simulink model "LunarMicrogrid_Full"  (R2026b)
settings: Solver=ode23t  StopTime=simulation.timeSim  MaxStep=1/(5*solarPlant.converterSwitchingFrequency)  AbsTol=1e-3
PreLoadFcn:
  | run('LunarMicrogridA_Data');
values from neighbouring files (symbols this model uses):
  Csc = Csc_cell/Ns_sc*Np_sc    (= 200)    [LunarDAB_Params.m]
  eta_sc = 0.95    [LunarDAB_Params.m]
  fsw = 100e3    (= 100000)    [LunarDAB_Params.m]
  k_restore = 1    [LunarDAB_Params.m]
  kiCurrent = 2    [LunarDAB_Params.m]
  kiVoltage = 8    [LunarDAB_Params.m]
  kpCurrent = 0.005    [LunarDAB_Params.m]
  kpVoltage = 0.4    [LunarDAB_Params.m]
  lTotal = lSeries + Llk    [LunarDAB_Params.m]
  P170_dt = 1e-4    (= 0.0001)    [P170_PV_Initialize.m]
  P170_Imp = im(ix)    [P170_PV_Initialize.m]
  P170_Vmp = vm(ix)    [P170_PV_Initialize.m]
  Rd_bat = dV_droop/Ibat_max    (= 0.232258064516)    [LunarDAB_Params.m]
  SC_enable = 1    [LunarDAB_Params.m]
  thetaIC = 0    [LunarDAB_Params.m]
  thetaMaxDab = pi/4    (= 0.785398163397)    [LunarDAB_Params.m]
  Tsw = 1/fsw    (= 1e-05)    [LunarDAB_Params.m]
  Vsc0 = sqrt((Vsc_max^2 + Vsc_min^2)/2)    [LunarDAB_Params.m]
  Vsc_max = 119    [LunarDAB_Params.m]
  Vsc_min = 66    [LunarDAB_Params.m]
undefined symbols (not defined in the file or in its folder): a_lpf_sys, battery, bms, connectedLoad, dcVoltage, DiscIntNeverNeededParam, eta_dab, Ibat_sign, mmc, Ndab, P170_T, pvDroop, sc, sensor, socLimit, solarPlant
libraries: sl_discontinuities x13, fl_lib x13, nesl_utility x13, simulink x7, batteryecm_lib x1, simulink_extras x1, ee_lib x1
(part 2 of 8)

== system LunarMicrogrid_Full/BESS Controller ==
  note: Current_Controller
  note: Voltage Controller
  Vref : Inport
  I_V1 : Inport  Port=2
  Vout : Inport  Port=3
  DABCtrl2 : Subsystem  AncestorBlock=mcblib/Control/Synchronous Machine/Controllers/PI Controller  mask(PID 1dof){Controller=PI, Form=Parallel, TimeDomain=Discrete-time, UseExternalTs=off, SampleTime=Tsw, IntegratorMethod=Forward Euler, FilterMethod=Forward Euler, ControllerParametersSource=internal, P=kpCurrent, I=kiCurrent, UseKiTs=off, D=0, UseExternalDerivativeSource=off, N=100, UseFilter=on, TunerSelectOption=Transfer Function Based (PID Tuner App), ZeroCross=on, InitialConditionSource=internal, InitialConditionForIntegrator=thetaIC, InitialConditionForFilter=0, DifferentiatorICPrevScaledInput=0, ExternalReset=none, IgnoreLimit=off, TrackingMode=off, Kt=1, LimitOutput=on, SatLimitsSource=external, UpperSaturationLimit=thetaMaxDab, LowerSaturationLimit=-thetaMaxDab, LinearizeAsGain=off, AntiWindupMode=clamping, Kb=1, LimitIntegrator=off, UpperIntegratorSaturationLimit=inf, LowerIntegratorSaturationLimit=-inf, RndMeth=Simplest, SaturateOnIntegerOverflow=off, LockScale=off, PGainOutDataTypeStr=Inherit: Same as input, PProdOutDataTypeStr=Inherit: Same as first input, POutMin=[], POutMax=[], IGainOutDataTypeStr=Inherit: Same as input, IProdOutDataTypeStr=Inherit: Same as first input, IOutMin=[], IOutMax=[], DGainOutDataTypeStr=Inherit: Inherit via internal rule, DProdOutDataTypeStr=Inherit: Inherit via internal rule, DOutMin=[], DOutMax=[], NGainOutDataTypeStr=Inherit: Inherit via internal rule, NProdOutDataTypeStr=Inherit: Inherit via internal rule, NOutMin=[], NOutMax=[], SumOutDataTypeStr=Inherit: Same as first input, SumOutMin=[], SumOutMax=[], SaturationOutDataTypeStr=Inherit: Inherit via back propagation, SaturationOutMin=[], SaturationOutMax=[], PParamDataTypeStr=Inherit: Inherit via internal rule, PParamMin=[], PParamMax=[], IParamDataTypeStr=Inherit: Inherit via internal rule, IParamMin=[], IParamMax=[], DParamDataTypeStr=Inherit: Inherit via internal rule, DParamMin=[], DParamMax=[], NParamDataTypeStr=Inherit: Inherit via internal rule, NParamMin=[], NParamMax=[], KbParamDataTypeStr=Inherit: Inherit via internal rule, KbParamMin=[], KbParamMax=[], KtParamDataTypeStr=Inherit: Inherit via internal rule, KtParamMin=[], KtParamMax=[], KbOutDataTypeStr=Inherit: Inherit via internal rule, KbOutMin=[], KbOutMax=[], KtOutDataTypeStr=Inherit: Inherit via internal rule, KtOutMin=[], KtOutMax=[], IntegratorOutDataTypeStr=Inherit: Inherit via internal rule, IntegratorOutMin=[], IntegratorOutMax=[], FilterOutDataTypeStr=Inherit: Inherit via internal rule, FilterOutMin=[], FilterOutMax=[], SumI1OutDataTypeStr=Inherit: Inherit via internal rule, SumI1OutMin=[], SumI1OutMax=[], SumI2OutDataTypeStr=Inherit: Inherit via internal rule, SumI2OutMin=[], SumI2OutMax=[], SumI3OutDataTypeStr=Inherit: Inherit via internal rule, SumI3OutMin=[], SumI3OutMax=[], SumI4OutDataTypeStr=Inherit: Inherit via internal rule, SumI4OutMin=[], SumI4OutMax=[], SumDOutDataTypeStr=Inherit: Inherit via internal rule, SumDOutMin=[], SumDOutMax=[], SumAccumDataTypeStr=Inherit: Inherit via internal rule, SumI1AccumDataTypeStr=Inherit: Inherit via internal rule, SumI2AccumDataTypeStr=Inherit: Inherit via internal rule, SumI3AccumDataTypeStr=Inherit: Inherit via internal rule, SumI4AccumDataTypeStr=Inherit: Inherit via internal rule, SumDAccumDataTypeStr=Inherit: Inherit via internal rule, DifferentiatorOutDataTypeStr=Inherit: Inherit via internal rule, DifferentiatorOutMin=[], DifferentiatorOutMax=[], FilterDiffNumProductOutputDataTypeStr=Inherit: Inherit via internal rule, FilterDiffDenProductOutputDataTypeStr=Inherit: Inherit via internal rule, FilterDiffNumAccumDataTypeStr=Inherit: Inherit via internal rule, FilterDiffDenAccumDataTypeStr=Inherit: Inherit via internal rule, FilterDiffOutCoefDataTypeStr=Inherit: Inherit via internal rule, FilterDiffOutCoefMin=[], FilterDiffOutCoefMax=[], ReciprocalOutDataTypeStr=Inherit: Inherit via internal rule, ReciprocalOutMin=[], ReciprocalOutMax=[], SumDenOutDataTypeStr=Inherit: Inherit via internal rule, SumDenOutMin=[], SumDenOutMax=[], SumNumOutDataTypeStr=Inherit: Inherit via internal rule, SumNumOutMin=[], SumNumOutMax=[], SumDenAccumDataTypeStr=Inherit: Inherit via internal rule, SumNumAccumDataTypeStr=Inherit: Inherit via internal rule, DivideOutDataTypeStr=Inherit: Inherit via internal rule, DivideOutMin=[], DivideOutMax=[], UdiffTsProdOutDataTypeStr=Inherit: Inherit via internal rule, UdiffTsProdOutMin=[], UdiffTsProdOutMax=[], NTsProdOutDataTypeStr=Inherit: Inherit via internal rule, NTsProdOutMin=[], NTsProdOutMax=[], UintegralTsProdOutDataTypeStr=Inherit: Inherit via internal rule, UintegralTsProdOutMin=[], UintegralTsProdOutMax=[], UngainTsProdOutDataTypeStr=Inherit: Inherit via internal rule, UngainTsProdOutMin=[], UngainTsProdOutMax=[], ClampingZeroOutDataTypeStr=Inherit: Inherit via back propagation, ClampingZeroOutMin=[], ClampingZeroOutMax=[], FilterDenConstantOutDataTypeStr=Inherit: Inherit via back propagation, FilterDenConstantOutMin=[], FilterDenConstantOutMax=[], PCopyOutDataTypeStr=Inherit: Inherit via back propagation, PCopyOutMin=[], PCopyOutMax=[], NCopyOutDataTypeStr=Inherit: Inherit via back propagation, NCopyOutMin=[], NCopyOutMax=[], IntegratorContinuousStateAttributes='', IntegratorStateIdentifier=, IntegratorStateMustResolveToSignalObject=off, IntegratorRTWStateStorageClass=Auto, IntegratorRTWStateStorageTypeQualifier=, FilterContinuousStateAttributes='', FilterStateIdentifier=, FilterStateMustResolveToSignalObject=off, FilterRTWStateStorageClass=Auto, FilterRTWStateStorageTypeQualifier=, ParallelPVariant=InternalParameters, IdealPVariant=Disabled, IVariant=InternalParameters, DVariant=Disabled, IntegratorVariant=Discrete, SatVariant=External, AWVariant=DiscClampingParallel, PCopyVariant=Disabled, TRVariant=Disabled, FdbkBlocksVariant=Forward, IdealPFdbkVariant=Disabled, SatFdbkVariant=Disabled, DerivativeFilterVariant=Disabled, NVariant=Disabled, NCopyVariant=Disabled_SignalSpec, FilterICVariant=Disabled, IntegratorICVariant=InternalICs, ExternalResetVariant=Disabled, TRSumVariant=Passthrough, SumFdbkVariant=Disabled, SumVariant=Sum_PI, TsampFilterVariant=InternalTs, TsampNgainVariant=Passthrough, TsampIntegralVariant=Disabled_SignalSpec, ExternalSaturationOutDataTypeStr=Inherit: Same as second input, DerivativeSourceVariant=Disabled, InitialConditionSetting=Auto, PreIntVariant=InternalPreInt}
      mask prompts: Controller "Simulink:masks:Controller_MP"; Form "Simulink:masks:Form_MP"; TimeDomain "Simulink:masks:TimeDomain_MP"; UseExternalTs "Simulink:masks:PIDBlockInTriggeredSubsystem_MP"; SampleTime "Simulink:masks:SampleTime1ForInherited_MP"; IntegratorMethod "Simulink:masks:IntegratorMethod_MP"; FilterMethod "Simulink:masks:FilterMethod_MP"; ControllerParametersSource "Simulink:masks:Source_MP"; P "Simulink:masks:ProportionalP_MP"; I "Simulink:masks:IntegralI_MP"; UseKiTs "Simulink:masks:UseITs_MP"; D "Simulink:masks:DerivativeD_MP"; UseExternalDerivativeSource "Simulink:masks:UseExternalDerivative_MP"; N "Simulink:masks:FilterCoefficientN_MP"; UseFilter "Simulink:masks:UseFilter_MP"; TunerSelectOption "Simulink:masks:PIDAutoTuningMethodSelect_MP"; ZeroCross "Simulink:masks:EnableZerocrossingDetection_MP"; InitialConditionSource "Simulink:masks:Source_MP"; InitialConditionForIntegrator "Simulink:masks:Integrator_MP"; InitialConditionForFilter "Simulink:masks:Filter_MP"; DifferentiatorICPrevScaledInput "Simulink:masks:Differentiator_MP"; ExternalReset "Simulink:masks:ExternalReset_MP"; IgnoreLimit "Simulink:masks:IgnoreResetWhenLinearizing_MP"; TrackingMode "Simulink:masks:EnableTrackingMode_MP"; Kt "Simulink:masks:TrackingCoefficientKt_MP"; LimitOutput "Simulink:masks:LimitOutput_MP"; SatLimitsSource "Simulink:masks:Source_MP"; UpperSaturationLimit "Simulink:masks:UpperSaturationLimit_MP"; LowerSaturationLimit "Simulink:masks:LowerSaturationLimit_MP"; LinearizeAsGain "Simulink:masks:IgnoreSaturationWhenLinearizing_MP"; AntiWindupMode "Simulink:masks:AntiwindupMethod_MP"; Kb "Simulink:masks:BackcalculationCoefficientKb_MP"; LimitIntegrator "Simulink:blkprm_prompts:IntegratorLimitOutput"; UpperIntegratorSaturationLimit "Simulink:masks:UpperSaturationLimit_MP"; LowerIntegratorSaturationLimit "Simulink:masks:LowerSaturationLimit_MP"; RndMeth "Simulink:masks:IntegerRoundingMode_MP"; SaturateOnIntegerOverflow "Simulink:masks:SaturateOnIntegerOverflow_MP"; LockScale "Simulink:masks:LockDataTypeAgainstFxpTools_MP"; PGainOutDataTypeStr "Simulink:masks:PProductOutput_MP"; PProdOutDataTypeStr "Simulink:masks:PProductOutput_MP"; IGainOutDataTypeStr "Simulink:masks:IProductOutput_MP"; IProdOutDataTypeStr "Simulink:masks:IProductOutput_MP"; DGainOutDataTypeStr "Simulink:masks:DProductOutput_MP"; DProdOutDataTypeStr "Simulink:masks:DProductOutput_MP"; NGainOutDataTypeStr "Simulink:masks:NProductOutput_MP"; NProdOutDataTypeStr "Simulink:masks:NProductOutput_MP"; SumOutDataTypeStr "Simulink:masks:SumOutput_MP"; SaturationOutDataTypeStr "Simulink:masks:SaturationOutput_MP"; PParamDataTypeStr "Simulink:masks:PParameter_MP"; IParamDataTypeStr "Simulink:masks:IParameter_MP"; DParamDataTypeStr "Simulink:masks:DParameter_MP"; NParamDataTypeStr "Simulink:masks:NParameter_MP"; KbParamDataTypeStr "Simulink:masks:KbParameter_MP"; KtParamDataTypeStr "Simulink:masks:KtParameter_MP"; KbOutDataTypeStr "Simulink:masks:KbProductOutput_MP"; KtOutDataTypeStr "Simulink:masks:KtProductOutput_MP"; IntegratorOutDataTypeStr "Simulink:masks:IntegratorOutput_MP"; FilterOutDataTypeStr "Simulink:masks:FilterOutput_MP"; SumI1OutDataTypeStr "Simulink:masks:SumI1Output_MP"; SumI2OutDataTypeStr "Simulink:masks:SumI2Output_MP"; SumI3OutDataTypeStr "Simulink:masks:SumI3Output_MP"; SumI4OutDataTypeStr "Simulink:masks:SumI4Output_MP"; SumDOutDataTypeStr "Simulink:masks:SumDOutput_MP"; SumAccumDataTypeStr "Simulink:masks:AccumulatorOfSum_MP"; SumI1AccumDataTypeStr "Simulink:masks:AccumulatorOfSumI1_MP"; SumI2AccumDataTypeStr "Simulink:masks:AccumulatorOfSumI2_MP"; SumI3AccumDataTypeStr "Simulink:masks:AccumulatorOfSumI3_MP"; SumI4AccumDataTypeStr "Simulink:masks:AccumulatorOfSumI4_MP"; SumDAccumDataTypeStr "Simulink:masks:AccumulatorOfSumD_MP"; DifferentiatorOutDataTypeStr "Simulink:masks:DifferentiatorOutput_MP"; FilterDiffNumProductOutputDataTypeStr "Simulink:masks:FilterDiffNumProductOutput_MP"; FilterDiffDenProductOutputDataTypeStr "Simulink:masks:FilterDiffDenProductOutput_MP"; FilterDiffNumAccumDataTypeStr "Simulink:masks:FilterDiffNumAccumulator_MP"; FilterDiffDenAccumDataTypeStr "Simulink:masks:FilterDiffDenAccumulator_MP"; FilterDiffOutCoefDataTypeStr "Simulink:masks:FilterDiffCoefficientOutput_MP"; ReciprocalOutDataTypeStr "Simulink:masks:FilterDiffReciprocalOutput_MP"; SumDenOutDataTypeStr "Simulink:masks:FilterDiffSumDenOutput_MP"; SumNumOutDataTypeStr "Simulink:masks:FilterDiffSumNumOutput_MP"; SumDenAccumDataTypeStr "Simulink:masks:FilterDiffSumDenAccumulator_MP"; SumNumAccumDataTypeStr "Simulink:masks:FilterDiffSumNumAccumulator_MP"; DivideOutDataTypeStr "Simulink:masks:FilterDiffDivideOutput_MP"; UdiffTsProdOutDataTypeStr "Simulink:masks:UdiffTsProdOut_MP"; NTsProdOutDataTypeStr "Simulink:masks:NTsProdOut_MP"; UintegralTsProdOutDataTypeStr "Simulink:masks:UintegralTsProdOut_MP"; UngainTsProdOutDataTypeStr "Simulink:masks:UngainTsProdOut_MP"; ClampingZeroOutDataTypeStr "Simulink:masks:ClampingAlgorithmConstantZero_MP"; FilterDenConstantOutDataTypeStr "Simulink:masks:FilterCoeffDenConstant_MP"; PCopyOutDataTypeStr "Simulink:masks:PCopyConstant_MP"; NCopyOutDataTypeStr "Simulink:masks:NCopyConstant_MP"; IntegratorContinuousStateAttributes "Simulink:masks:StateNameegposition_MP"; IntegratorStateIdentifier "Simulink:masks:StateName_MP"; IntegratorStateMustResolveToSignalObject "Simulink:masks:StateNameMustResolveToSimulinkSignalObject_MP"; IntegratorRTWStateStorageClass "Simulink:masks:CodeGenerationStorageClass_MP"; IntegratorRTWStateStorageTypeQualifier "Simulink:masks:CodeGenerationStorageTypeQualifier_MP"; FilterContinuousStateAttributes "Simulink:masks:StateNameegposition_MP"; FilterStateIdentifier "Simulink:masks:StateName_MP"; FilterStateMustResolveToSignalObject "Simulink:masks:StateNameMustResolveToSimulinkSignalObject_MP"; FilterRTWStateStorageClass "Simulink:masks:CodeGenerationStorageClass_MP"; FilterRTWStateStorageTypeQualifier "Simulink:masks:CodeGenerationStorageTypeQualifier_MP"; ParallelPVariant "Simulink:blkprm_prompts:OverrideUsingVariant"; IdealPVariant "Simulink:blkprm_prompts:OverrideUsingVariant"; IVariant "Simulink:blkprm_prompts:OverrideUsingVariant"; DVariant "Simulink:blkprm_prompts:OverrideUsingVariant"; IntegratorVariant "Simulink:blkprm_prompts:OverrideUsingVariant"; SatVariant "Simulink:blkprm_prompts:OverrideUsingVariant"; AWVariant "Simulink:blkprm_prompts:OverrideUsingVariant"; PCopyVariant "Simulink:blkprm_prompts:OverrideUsingVariant"; TRVariant "Simulink:blkprm_prompts:OverrideUsingVariant"; FdbkBlocksVariant "Simulink:blkprm_prompts:OverrideUsingVariant"; IdealPFdbkVariant "Simulink:blkprm_prompts:OverrideUsingVariant"; SatFdbkVariant "Simulink:blkprm_prompts:OverrideUsingVariant"; DerivativeFilterVariant "Simulink:blkprm_prompts:OverrideUsingVariant"; NVariant "Simulink:blkprm_prompts:OverrideUsingVariant"; NCopyVariant "Simulink:blkprm_prompts:OverrideUsingVariant"; FilterICVariant "Simulink:blkprm_prompts:OverrideUsingVariant"; IntegratorICVariant "Simulink:blkprm_prompts:OverrideUsingVariant"; ExternalResetVariant "Simulink:blkprm_prompts:OverrideUsingVariant"; TRSumVariant "Simulink:blkprm_prompts:OverrideUsingVariant"; SumFdbkVariant "Simulink:blkprm_prompts:OverrideUsingVariant"; SumVariant "Simulink:blkprm_prompts:OverrideUsingVariant"; TsampFilterVariant "Simulink:Variants:LabelComboBox"; TsampNgainVariant "Simulink:Variants:LabelComboBox"; TsampIntegralVariant "Simulink:Variants:LabelComboBox"; ExternalSaturationOutDataTypeStr "Simulink:masks:SaturationOutput_MP"; DerivativeSourceVariant "Simulink:Variants:LabelComboBox"; InitialConditionSetting "Simulink:blkprm_prompts:IntegratorInitCondSetting"; PreIntVariant "Simulink:Variants:LabelComboBox"
      mask help: Simulink:masks:PID1dof_MD
      mask init:
      | SampleTime = pidpack.PIDConfig.maskInitialization(gcbh, SampleTime);
      settings: LibrarySourceBlock=mcblib/Control/Synchronous Machine/Controllers/PI Controller  DeleteFcn=pidpack.PIDConfig.utilCloseTuner(gcb)  ModelCloseFcn=pidpack.PIDConfig.utilCloseTuner(gcb)  NameChangeFcn=pidpack.PIDConfig.utilUpdateTunerName(gcb)
      mask TypeOptions Controller: Simulink:masks:PID | Simulink:masks:PI | Simulink:masks:PD | Simulink:masks:P | Simulink:masks:I
      mask Callback Controller: pidpack.PIDConfig.callbackMaskVisibilities(gcbh,'UpdateCompFormula')
      mask TypeOptions Form: Simulink:masks:Ideal | Simulink:masks:Parallel
      mask Callback Form: pidpack.PIDConfig.callbackMaskVisibilities(gcbh,'UpdateCompFormula')
      mask TypeOptions TimeDomain: Simulink:masks:ContinuousTime | Simulink:masks:DiscreteTime
      mask Callback TimeDomain: pidpack.PIDConfig.callbackMaskVisibilities(gcbh,'UpdateCompFormula')
      mask Callback UseExternalTs: pidpack.PIDConfig.callbackMaskVisibilities(gcbh)
      mask TypeOptions SampleTime: u/SampleTime | Anti-windup/preSat/SampleTime | Anti-windup/postSat/SampleTime | Anti-windup/P/SampleTime | Anti-windup/preInt/SampleTime | Anti-windup/Back Calculation/preSat/SampleTime | Anti-windup/Back Calculation/postSat/SampleTime | Anti-windup/Back Calculation/preInt/SampleTime | Anti-windup/Back Calculation/Out1/SampleTime | Anti-windup/Cont. Clamping Ideal/preSat/SampleTime | Anti-windup/Cont. Clamping Ideal/P/SampleTime | Anti-windup/Cont. Clamping Ideal/preInt/SampleTime | Anti-windup/Cont. Clamping Ideal/Out1/SampleTime | Anti-windup/Disc. Clamping Parallel/preSat/SampleTime | Anti-windup/Disc. Clamping Parallel/preInt/SampleTime | Anti-windup/Disc. Clamping Parallel/Out1/SampleTime | Anti-windup/Passthrough/Out1/SampleTime | Anti-windup/Out1/SampleTime | D Gain/err/SampleTime | D Gain/D Gain/SampleTime | D Gain/External Parameters/err/SampleTime | D Gain/External Parameters/D Gain/SampleTime | D Gain/External Parameters/DProd Out/SampleTime | D Gain/External Parameters/Out1/SampleTime | D Gain/Internal Parameters/err/SampleTime | D Gain/Internal Parameters/Out1/SampleTime | D Gain/Out1/SampleTime | Filter/Reset/SampleTime | Filter/U/SampleTime | Filter/N/SampleTime | Filter/D0in/SampleTime | Filter/Nout/SampleTime | Filter/Cont. Filter/U/SampleTime | Filter/Cont. Filter/Nout/SampleTime | Filter/Cont. Filter/Reset/SampleTime | Filter/Cont. Filter/D0in/SampleTime | Filter/Cont. Filter/Y/SampleTime | Filter/Differentiator/U/SampleTime | Filter/Differentiator/Reset/SampleTime | Filter/Differentiator/D0in/SampleTime | Filter/Differentiator/UD/SampleTime | Filter/Differentiator/Y/SampleTime | Filter/Disc. Backward Euler Filter/U/SampleTime | Filter/Disc. Backward Euler Filter/N/SampleTime | Filter/Disc. Backward Euler Filter/Reset/SampleTime | Filter/Disc. Backward Euler Filter/D0in/SampleTime | Filter/Disc. Backward Euler Filter/DenCoefOut/SampleTime | Filter/Disc. Backward Euler Filter/Filter Differentiator TF/SampleTime | Filter/Disc. Backward Euler Filter/Y/SampleTime | Filter/Disc. Forward Euler Filter/U/SampleTime | Filter/Disc. Forward Euler Filter/Nout/SampleTime | Filter/Disc. Forward Euler Filter/Reset/SampleTime | Filter/Disc. Forward Euler Filter/D0in/SampleTime | Filter/Disc. Forward Euler Filter/Filter/SampleTime | Filter/Disc. Forward Euler Filter/Y/SampleTime | Filter/Disc. Trapezoidal Filter/U/SampleTime | Filter/Disc. Trapezoidal Filter/N/SampleTime | Filter/Disc. Trapezoidal Filter/Reset/SampleTime | Filter/Disc. Trapezoidal Filter/D0in/SampleTime | Filter/Disc. Trapezoidal Filter/DenCoefOut/SampleTime | Filter/Disc. Trapezoidal Filter/Divide/SampleTime | Filter/Disc. Trapezoidal Filter/Filter Differentiator TF/SampleTime | Filter/Disc. Trapezoidal Filter/Y/SampleTime | Filter/Y/SampleTime | Filter ICs/D0/SampleTime | Filter ICs/External IC/D0/SampleTime | Filter ICs/External IC/Out1/SampleTime | Filter ICs/Internal IC - Differentiator/Out1/SampleTime | Filter ICs/Internal IC - Filter/Out1/SampleTime | Filter ICs/Out1/SampleTime | I Gain/err/SampleTime | I Gain/I Gain/SampleTime | I Gain/External Parameters/err/SampleTime | I Gain/External Parameters/I Gain/SampleTime | I Gain/External Parameters/IProd Out/SampleTime | I Gain/External Parameters/Out1/SampleTime | I Gain/Internal Parameters/err/SampleTime | I Gain/Internal Parameters/Out1/SampleTime | I Gain/Out1/SampleTime | Ideal P Gain/In1/SampleTime | Ideal P Gain/P Gain/SampleTime | Ideal P Gain/External Parameters/In1/SampleTime | Ideal P Gain/External Parameters/P Gain/SampleTime | Ideal P Gain/External Parameters/PProd Out/SampleTime | Ideal P Gain/External Parameters/Out1/SampleTime | Ideal P Gain/Internal Parameters/In1/SampleTime | Ideal P Gain/Internal Parameters/Out1/SampleTime | Ideal P Gain/Passthrough/In1/SampleTime | Ideal P Gain/Passthrough/Out1/SampleTime | Ideal P Gain/Out1/SampleTime | Ideal P Gain Fdbk/In1/SampleTime | Ideal P Gain Fdbk/P Gain/SampleTime | Ideal P Gain Fdbk/External Parameters/In1/SampleTime | Ideal P Gain Fdbk/External Parameters/P Gain/SampleTime | Ideal P Gain Fdbk/External Parameters/PProd Out/SampleTime | Ideal P Gain Fdbk/External Parameters/Out1/SampleTime | Ideal P Gain Fdbk/Internal Parameters/In1/SampleTime | Ideal P Gain Fdbk/Internal Parameters/Out1/SampleTime | Ideal P Gain Fdbk/Passthrough/In1/SampleTime | Ideal P Gain Fdbk/Passthrough/Out1/SampleTime | Ideal P Gain Fdbk/Out1/SampleTime | Integrator/U/SampleTime | Integrator/I0in/SampleTime | Integrator/Reset/SampleTime | Integrator/Continuous/U/SampleTime | Integrator/Continuous/Reset/SampleTime | Integrator/Continuous/I0in/SampleTime | Integrator/Continuous/out/SampleTime | Integrator/Discrete/U/SampleTime | Integrator/Discrete/Reset/SampleTime | Integrator/Discrete/I0in/SampleTime | Integrator/Discrete/Integrator/SampleTime | Integrator/Discrete/out/SampleTime | Integrator/Discrete/state/SampleTime | Integrator/state/SampleTime | Integrator/out/SampleTime | Integrator ICs/I0/SampleTime | Integrator ICs/External IC/I0/SampleTime | Integrator ICs/External IC/Out1/SampleTime | Integrator ICs/Internal IC/Out1/SampleTime | Integrator ICs/Out1/SampleTime | N Copy/N Gain/SampleTime | N Copy/External Parameters/N Gain/SampleTime | N Copy/External Parameters/Out1/SampleTime | N Copy/Internal Parameters/Out1/SampleTime | N Copy/Out1/SampleTime | N Gain/U/SampleTime | N Gain/N Gain/SampleTime | N Gain/External Parameters/U/SampleTime | N Gain/External Parameters/N Gain/SampleTime | N Gain/External Parameters/NProd Out/SampleTime | N Gain/External Parameters/Out1/SampleTime | N Gain/Internal Parameters/U/SampleTime | N Gain/Internal Parameters/Out1/SampleTime | N Gain/Passthrough/U/SampleTime | N Gain/Passthrough/Out1/SampleTime | N Gain/Out1/SampleTime | P Copy/P Gain/SampleTime | P Copy/External Parameters Ideal/P Gain/SampleTime | P Copy/External Parameters Ideal/Out1/SampleTime | P Copy/Internal Parameters Ideal/Out1/SampleTime | P Copy/Out1/SampleTime | Parallel P Gain/err/SampleTime | Parallel P Gain/P Gain/SampleTime | Parallel P Gain/External Parameters/err/SampleTime | Parallel P Gain/External Parameters/P Gain/SampleTime | Parallel P Gain/External Parameters/PProd Out/SampleTime | Parallel P Gain/External Parameters/Out1/SampleTime | Parallel P Gain/Internal Parameters/err/SampleTime | Parallel P Gain/Internal Parameters/Out1/SampleTime | Parallel P Gain/Passthrough/err/SampleTime | Parallel P Gain/Passthrough/Out1/SampleTime | Parallel P Gain/Out1/SampleTime | Saturation/In1/SampleTime | Saturation/Enabled/In1/SampleTime | Saturation/Enabled/Saturation/SampleTime | Saturation/Enabled/Out1/SampleTime | Saturation/Passthrough/In1/SampleTime | Saturation/Passthrough/Out1/SampleTime | Saturation/Out1/SampleTime | Saturation Fdbk/In1/SampleTime | Saturation Fdbk/Enabled/In1/SampleTime | Saturation Fdbk/Enabled/Saturation/SampleTime | Saturation Fdbk/Enabled/Out1/SampleTime | Saturation Fdbk/Passthrough/In1/SampleTime | Saturation Fdbk/Passthrough/Out1/SampleTime | Saturation Fdbk/Out1/SampleTime | Tracking Mode/uout/SampleTime | Tracking Mode/TR/SampleTime | Tracking Mode/Enabled/uout/SampleTime | Tracking Mode/Enabled/TR/SampleTime | Tracking Mode/Enabled/Out1/SampleTime | Tracking Mode/Out1/SampleTime | postSat Signal/feedback/SampleTime | postSat Signal/forward/SampleTime | postSat Signal/Feedback_Path/feedback/SampleTime | postSat Signal/Feedback_Path/Out1/SampleTime | postSat Signal/Forward_Path/forward/SampleTime | postSat Signal/Forward_Path/Out1/SampleTime | postSat Signal/Out1/SampleTime | preSat Signal/feedback/SampleTime | preSat Signal/forward/SampleTime | preSat Signal/Feedback_Path/feedback/SampleTime | preSat Signal/Feedback_Path/Out1/SampleTime | preSat Signal/Forward_Path/forward/SampleTime | preSat Signal/Forward_Path/Out1/SampleTime | preSat Signal/Out1/SampleTime | Anti-windup/Disc. Clamping Parallel/Switch/SampleTime | Anti-windup/Cont. Clamping Parallel/preSat/SampleTime | Anti-windup/Cont. Clamping Parallel/preInt/SampleTime | Anti-windup/Cont. Clamping Parallel/Out1/SampleTime | Anti-windup/Disc. Clamping Ideal/preSat/SampleTime | Anti-windup/Disc. Clamping Ideal/P/SampleTime | Anti-windup/Disc. Clamping Ideal/preInt/SampleTime | Anti-windup/Disc. Clamping Ideal/Out1/SampleTime | Reset Signal/Reset/SampleTime | Reset Signal/External Reset/Reset/SampleTime | Reset Signal/External Reset/Out1/SampleTime | Reset Signal/Out1/SampleTime | Anti-windup/Disabled/preInt/SampleTime | Anti-windup/Back Calculation/P/SampleTime | Anti-windup/Back Calculation/Signal Specification2/SampleTime | Anti-windup/Cont. Clamping Ideal/postSat/SampleTime | Anti-windup/Cont. Clamping Parallel/postSat/SampleTime | Anti-windup/Cont. Clamping Parallel/P/SampleTime | Anti-windup/Cont. Clamping Parallel/Signal Specification2/SampleTime | Anti-windup/Disabled/preSat/SampleTime | Anti-windup/Disabled/postSat/SampleTime | Anti-windup/Disabled/P/SampleTime | Anti-windup/Disabled/Signal Specification1/SampleTime | Anti-windup/Disabled/Signal Specification2/SampleTime | Anti-windup/Disc. Clamping Ideal/postSat/SampleTime | Anti-windup/Disc. Clamping Parallel/postSat/SampleTime | Anti-windup/Disc. Clamping Parallel/P/SampleTime | Anti-windup/Disc. Clamping Parallel/Signal Specification2/SampleTime | Anti-windup/Passthrough/preInt/SampleTime | Anti-windup/Passthrough/preSat/SampleTime | Anti-windup/Passthrough/postSat/SampleTime | Anti-windup/Passthrough/P/SampleTime | Anti-windup/Passthrough/Signal Specification2/SampleTime | D Gain/Disabled/D Gain/SampleTime | D Gain/Disabled/Signal Specification/SampleTime | D Gain/Internal Parameters/D Gain/SampleTime | D Gain/Internal Parameters/Signal Specification/SampleTime | Filter/Cont. Filter/N/SampleTime | Filter/Cont. Filter/Signal Specification2/SampleTime | Filter/Differentiator/Nout/SampleTime | Filter/Differentiator/N/SampleTime | Filter/Differentiator/Signal Specification1/SampleTime | Filter/Disabled/Reset/SampleTime | Filter/Disabled/U/SampleTime | Filter/Disabled/N/SampleTime | Filter/Disabled/D0in/SampleTime | Filter/Disabled/Nout/SampleTime | Filter/Disabled/Signal Specification1/SampleTime | Filter/Disabled/Signal Specification2/SampleTime | Filter/Disabled/Signal Specification3/SampleTime | Filter/Disabled/Signal Specification4/SampleTime | Filter/Disc. Backward Euler Filter/Nout/SampleTime | Filter/Disc. Forward Euler Filter/N/SampleTime | Filter/Disc. Forward Euler Filter/Signal Specification2/SampleTime | Filter/Disc. Trapezoidal Filter/Nout/SampleTime | Filter ICs/Disabled/D0/SampleTime | Filter ICs/Disabled/Signal Specification/SampleTime | Filter ICs/Disabled/Signal Specification1/SampleTime | Filter ICs/Disabled/Out1/SampleTime | Filter ICs/Internal IC - Differentiator/D0/SampleTime | Filter ICs/Internal IC - Differentiator/Signal Specification/SampleTime | Filter ICs/Internal IC - Differentiator/Signal Specification1/SampleTime | Filter ICs/Internal IC - Filter/D0/SampleTime | Filter ICs/Internal IC - Filter/Signal Specification/SampleTime | Filter ICs/Internal IC - Filter/Signal Specification1/SampleTime | I Gain/Disabled/I Gain/SampleTime | I Gain/Disabled/Signal Specification/SampleTime | I Gain/Internal Parameters/I Gain/SampleTime | I Gain/Internal Parameters/Signal Specification/SampleTime | Ideal P Gain/Internal Parameters/P Gain/SampleTime | Ideal P Gain/Internal Parameters/Signal Specification1/SampleTime | Ideal P Gain/Passthrough/P Gain/SampleTime | Ideal P Gain Fdbk/Disabled/In1/SampleTime | Ideal P Gain Fdbk/Disabled/P Gain/SampleTime | Ideal P Gain Fdbk/Disabled/Signal Specification1/SampleTime | Ideal P Gain Fdbk/Internal Parameters/P Gain/SampleTime | Ideal P Gain Fdbk/Internal Parameters/Signal Specification1/SampleTime | Ideal P Gain Fdbk/Passthrough/P Gain/SampleTime | Integrator/Continuous/Signal Specification1/SampleTime | Integrator/Continuous/state/SampleTime | Integrator/Disabled/U/SampleTime | Integrator/Disabled/Reset/SampleTime | Integrator/Disabled/I0in/SampleTime | Integrator/Disabled/Signal Specification1/SampleTime | Integrator/Disabled/Signal Specification2/SampleTime | Integrator/Disabled/Signal Specification4/SampleTime | Integrator/Disabled/out/SampleTime | Integrator/Discrete/Signal Specification1/SampleTime | Integrator ICs/Disabled/I0/SampleTime | Integrator ICs/Disabled/Signal Specification/SampleTime | Integrator ICs/Disabled/Signal Specification1/SampleTime | Integrator ICs/Disabled/Out1/SampleTime | Integrator ICs/Internal IC/I0/SampleTime | Integrator ICs/Internal IC/Signal Specification/SampleTime | Integrator ICs/Internal IC/Signal Specification1/SampleTime | N Copy/Disabled/N Gain/SampleTime | N Copy/Disabled wSignal Specification/N Gain/SampleTime | N Copy/Disabled wSignal Specification/Signal Specification1/SampleTime | N Copy/Internal Parameters/N Gain/SampleTime | N Copy/Internal Parameters/Signal Specification/SampleTime | N Gain/Disabled/U/SampleTime | N Gain/Disabled/N Gain/SampleTime | N Gain/Disabled/Signal Specification1/SampleTime | N Gain/Disabled/Signal Specification2/SampleTime | N Gain/Internal Parameters/N Gain/SampleTime | N Gain/Internal Parameters/Signal Specification1/SampleTime | N Gain/Passthrough/N Gain/SampleTime | P Copy/Disabled/P Gain/SampleTime | P Copy/Internal Parameters Ideal/P Gain/SampleTime | Parallel P Gain/Disabled/P Gain/SampleTime | Parallel P Gain/Disabled/Signal Specification/SampleTime | Parallel P Gain/Internal Parameters/P Gain/SampleTime | Parallel P Gain/Internal Parameters/Signal Specification/SampleTime | Parallel P Gain/Passthrough/P Gain/SampleTime | Reset Signal/Disabled/Reset/SampleTime | Reset Signal/Disabled/Signal Specification/SampleTime | Reset Signal/Disabled/Signal Specification1/SampleTime | Reset Signal/Disabled/Out1/SampleTime | Saturation Fdbk/Disabled/In1/SampleTime | Saturation Fdbk/Disabled/Signal Specification1/SampleTime | Sum/P/SampleTime | Sum/I/SampleTime | Sum/D/SampleTime | Sum/Passthrough_I/I/SampleTime | Sum/Passthrough_I/Out1/SampleTime | Sum/Passthrough_P/P/SampleTime | Sum/Passthrough_P/Out1/SampleTime | Sum/Sum_PD/P/SampleTime | Sum/Sum_PD/D/SampleTime | Sum/Sum_PD/Out1/SampleTime | Sum/Sum_PI/P/SampleTime | Sum/Sum_PI/I/SampleTime | Sum/Sum_PI/Out1/SampleTime | Sum/Sum_PID/P/SampleTime | Sum/Sum_PID/I/SampleTime | Sum/Sum_PID/D/SampleTime | Sum/Sum_PID/Out1/SampleTime | Sum/Out1/SampleTime | Sum Fdbk/fromP/SampleTime | Sum Fdbk/fromState/SampleTime | Sum Fdbk/fromD/SampleTime | Sum Fdbk/Disabled/fromP/SampleTime | Sum Fdbk/Disabled/fromState/SampleTime | Sum Fdbk/Disabled/fromD/SampleTime | Sum Fdbk/Disabled/Signal Specification1/SampleTime | Sum Fdbk/Enabled/fromP/SampleTime | Sum Fdbk/Enabled/fromState/SampleTime | Sum Fdbk/Enabled/fromD/SampleTime | Sum Fdbk/Enabled/Out1/SampleTime | Sum Fdbk/Passthrough/fromState/SampleTime | Sum Fdbk/Passthrough/Out1/SampleTime | Sum Fdbk/Out1/SampleTime | Tracking Mode/Disabled/uout/SampleTime | Tracking Mode/Disabled/TR/SampleTime | Tracking Mode/Disabled/Signal Specification1/SampleTime | Tracking Mode Sum/fromIgain/SampleTime | Tracking Mode Sum/fromTR/SampleTime | Tracking Mode Sum/Passthrough/fromIgain/SampleTime | Tracking Mode Sum/Passthrough/fromTR/SampleTime | Tracking Mode Sum/Passthrough/Signal Specification/SampleTime | Tracking Mode Sum/Passthrough/Out1/SampleTime | Tracking Mode Sum/Tracking Mode/fromIgain/SampleTime | Tracking Mode Sum/Tracking Mode/fromTR/SampleTime | Tracking Mode Sum/Tracking Mode/Out1/SampleTime | Tracking Mode Sum/Out1/SampleTime | postSat Signal/Feedback_Path/forward/SampleTime | postSat Signal/Forward_Path/feedback/SampleTime | postSat Signal/Forward_Path/Signal Specification1/SampleTime | preSat Signal/Feedback_Path/forward/SampleTime | preSat Signal/Forward_Path/feedback/SampleTime | preSat Signal/Forward_Path/Signal Specification1/SampleTime | Filter/Ts/SampleTime | Filter/Cont. Filter/Ts/SampleTime | Filter/Differentiator/Ts/SampleTime | Filter/Differentiator/Tsamp/U/SampleTime | Filter/Differentiator/Tsamp/Ts/SampleTime | Filter/Differentiator/Tsamp/External Ts/U/SampleTime | Filter/Differentiator/Tsamp/External Ts/Ts/SampleTime | Filter/Differentiator/Tsamp/External Ts/Udiff*Ts Prod Out/SampleTime | Filter/Differentiator/Tsamp/External Ts/Out1/SampleTime | Filter/Differentiator/Tsamp/Internal Ts/U/SampleTime | Filter/Differentiator/Tsamp/Internal Ts/Ts/SampleTime | Filter/Differentiator/Tsamp/Internal Ts/Out1/SampleTime | Filter/Differentiator/Tsamp/Out1/SampleTime | Filter/Disabled/Ts/SampleTime | Filter/Disc. Backward Euler Filter/Ts/SampleTime | Filter/Disc. Backward Euler Filter/Tsamp/N/SampleTime | Filter/Disc. Backward Euler Filter/Tsamp/Ts/SampleTime | Filter/Disc. Backward Euler Filter/Tsamp/External Ts/N/SampleTime | Filter/Disc. Backward Euler Filter/Tsamp/External Ts/Ts/SampleTime | Filter/Disc. Backward Euler Filter/Tsamp/External Ts/N*Ts Prod Out/SampleTime | Filter/Disc. Backward Euler Filter/Tsamp/External Ts/Out1/SampleTime | Filter/Disc. Backward Euler Filter/Tsamp/Internal Ts/N/SampleTime | Filter/Disc. Backward Euler Filter/Tsamp/Internal Ts/Ts/SampleTime | Filter/Disc. Backward Euler Filter/Tsamp/Internal Ts/Out1/SampleTime | Filter/Disc. Backward Euler Filter/Tsamp/Out1/SampleTime | Filter/Disc. Forward Euler Filter/Ts/SampleTime | Filter/Disc. Trapezoidal Filter/Ts/SampleTime | Filter/Disc. Trapezoidal Filter/Tsamp/N/SampleTime | Filter/Disc. Trapezoidal Filter/Tsamp/Ts/SampleTime | Filter/Disc. Trapezoidal Filter/Tsamp/External Ts/N/SampleTime | Filter/Disc. Trapezoidal Filter/Tsamp/External Ts/Ts/SampleTime | Filter/Disc. Trapezoidal Filter/Tsamp/External Ts/N*Ts Prod Out/SampleTime | Filter/Disc. Trapezoidal Filter/Tsamp/External Ts/Out1/SampleTime | Filter/Disc. Trapezoidal Filter/Tsamp/Internal Ts/N/SampleTime | Filter/Disc. Trapezoidal Filter/Tsamp/Internal Ts/Ts/SampleTime | Filter/Disc. Trapezoidal Filter/Tsamp/Internal Ts/Out1/SampleTime | Filter/Disc. Trapezoidal Filter/Tsamp/Out1/SampleTime | Tsamp - Integral/U/SampleTime | Tsamp - Integral/Ts/SampleTime | Tsamp - Integral/Disabled/U/SampleTime | Tsamp - Integral/Disabled/Ts/SampleTime | Tsamp - Integral/Disabled/Out1/SampleTime | Tsamp - Integral/Disabled wSignal Specification/U/SampleTime | Tsamp - Integral/Disabled wSignal Specification/Ts/SampleTime | Tsamp - Integral/Disabled wSignal Specification/Signal Specification/SampleTime | Tsamp - Integral/Disabled wSignal Specification/Out1/SampleTime | Tsamp - Integral/External Ts/U/SampleTime | Tsamp - Integral/External Ts/Ts/SampleTime | Tsamp - Integral/External Ts/Uintegral*Ts Prod Out/SampleTime | Tsamp - Integral/External Ts/Out1/SampleTime | Tsamp - Integral/Passthrough/U/SampleTime | Tsamp - Integral/Passthrough/Ts/SampleTime | Tsamp - Integral/Passthrough/Signal Specification/SampleTime | Tsamp - Integral/Passthrough/Out1/SampleTime | Tsamp - Integral/Out1/SampleTime | Tsamp - Ngain/U/SampleTime | Tsamp - Ngain/Ts/SampleTime | Tsamp - Ngain/External Ts/U/SampleTime | Tsamp - Ngain/External Ts/Ts/SampleTime | Tsamp - Ngain/External Ts/Ungain*Ts Prod Out/SampleTime | Tsamp - Ngain/External Ts/Out1/SampleTime | Tsamp - Ngain/Passthrough/U/SampleTime | Tsamp - Ngain/Passthrough/Ts/SampleTime | Tsamp - Ngain/Passthrough/Out1/SampleTime | Tsamp - Ngain/Out1/SampleTime | y/SampleTime
      mask TypeOptions IntegratorMethod: Simulink:masks:ForwardEuler | Simulink:masks:BackwardEuler | Simulink:masks:Trapezoidal
      mask Callback IntegratorMethod: pidpack.PIDConfig.callbackMaskVisibilities(gcbh,'UpdateCompFormula')
      mask TypeOptions FilterMethod: Simulink:masks:ForwardEuler | Simulink:masks:BackwardEuler | Simulink:masks:Trapezoidal
      mask Callback FilterMethod: pidpack.PIDConfig.callbackMaskVisibilities(gcbh,'UpdateCompFormula')
      mask TypeOptions ControllerParametersSource: Simulink:masks:internal | Simulink:masks:external
      mask Callback ControllerParametersSource: pidpack.PIDConfig.callbackMaskVisibilities(gcbh)
      mask TypeOptions P: Parallel P Gain/Internal Parameters/Proportional Gain/Gain | P Copy/Internal Parameters Ideal/P Copy/Value | Ideal P Gain/Internal Parameters/Proportional Gain/Gain | Ideal P Gain Fdbk/Internal Parameters/Proportional Gain/Gain
      mask TypeOptions I: I Gain/Internal Parameters/Integral Gain/Gain
      mask Callback UseKiTs: pidpack.PIDConfig.callbackIntegralType(gcbh)
      mask TypeOptions D: D Gain/Internal Parameters/Derivative Gain/Gain
      mask TypeOptions N: N Gain/Internal Parameters/Filter Coefficient/Gain | N Copy/Internal Parameters/N Copy/Value
      mask Callback UseFilter: pidpack.PIDConfig.callbackMaskVisibilities(gcbh,'UpdateCompFormula')
      mask TypeOptions TunerSelectOption: Simulink:masks:UsePIDTunerApp | Simulink:masks:UseOLSimulation
      mask Callback TunerSelectOption: pidpack.PIDConfig.callbackTunerSelect(gcbh)
      mask TypeOptions ZeroCross: Integrator/Continuous/Integrator/ZeroCross | Anti-windup/Cont. Clamping Ideal/Equal1/ZeroCross | Anti-windup/Cont. Clamping Ideal/Equal2/ZeroCross | Anti-windup/Cont. Clamping Ideal/NotEqual/ZeroCross | Anti-windup/Cont. Clamping Ideal/SignP/ZeroCross | Anti-windup/Cont. Clamping Ideal/SignPreIntegrator/ZeroCross | Anti-windup/Cont. Clamping Ideal/SignPreSat/ZeroCross | Anti-windup/Cont. Clamping Ideal/Switch/ZeroCross | Anti-windup/Disc. Clamping Parallel/Equal1/ZeroCross | Anti-windup/Disc. Clamping Parallel/NotEqual/ZeroCross | Anti-windup/Disc. Clamping Parallel/SignPreIntegrator/ZeroCross | Anti-windup/Disc. Clamping Parallel/SignPreSat/ZeroCross | Anti-windup/Disc. Clamping Parallel/Switch/ZeroCross | Filter/Cont. Filter/Filter/ZeroCross | Saturation/Enabled/Saturation/ZeroCross | Saturation Fdbk/Enabled/Saturation/ZeroCross | Anti-windup/Cont. Clamping Parallel/Equal1/ZeroCross | Anti-windup/Cont. Clamping Parallel/NotEqual/ZeroCross | Anti-windup/Cont. Clamping Parallel/SignPreIntegrator/ZeroCross | Anti-windup/Cont. Clamping Parallel/SignPreSat/ZeroCross | Anti-windup/Cont. Clamping Parallel/Switch/ZeroCross | Anti-windup/Disc. Clamping Ideal/Equal1/ZeroCross | Anti-windup/Disc. Clamping Ideal/Equal2/ZeroCross | Anti-windup/Disc. Clamping Ideal/NotEqual/ZeroCross | Anti-windup/Disc. Clamping Ideal/SignP/ZeroCross | Anti-windup/Disc. Clamping Ideal/SignPreIntegrator/ZeroCross | Anti-windup/Disc. Clamping Ideal/SignPreSat/ZeroCross | Anti-windup/Disc. Clamping Ideal/Switch/ZeroCross | Anti-windup/Cont. Clamping Ideal/Dead Zone/Enabled/DeadZone/ZeroCross | Anti-windup/Cont. Clamping Parallel/Dead Zone/Enabled/DeadZone/ZeroCross | Anti-windup/Disc. Clamping Ideal/Dead Zone/Enabled/DeadZone/ZeroCross | Anti-windup/Disc. Clamping Parallel/Dead Zone/Enabled/DeadZone/ZeroCross
      mask TypeOptions InitialConditionSource: Simulink:masks:internal | Simulink:masks:external
      mask Callback InitialConditionSource: pidpack.PIDConfig.callbackMaskVisibilities(gcbh)
      mask TypeOptions DifferentiatorICPrevScaledInput: Filter/Differentiator/UD/InitialCondition
      mask TypeOptions ExternalReset: Simulink:masks:none | Simulink:masks:rising | Simulink:masks:falling | Simulink:masks:either | Simulink:masks:level
      mask TypeOptions IgnoreLimit: Integrator/Continuous/Integrator/IgnoreLimit | Filter/Cont. Filter/Filter/IgnoreLimit | Filter/Disc. Forward Euler Filter/Filter/IgnoreLimit | Integrator/Discrete/Integrator/IgnoreLimit
      mask Callback TrackingMode: pidpack.PIDConfig.callbackMaskVisibilities(gcbh)
      mask TypeOptions Kt: Tracking Mode/Enabled/Kt/Gain
      mask Callback LimitOutput: pidpack.PIDConfig.callbackMaskVisibilities(gcbh)
      mask TypeOptions SatLimitsSource: Simulink:masks:internal | Simulink:masks:external
      mask Callback SatLimitsSource: pidpack.PIDConfig.callbackMaskVisibilities(gcbh)
      mask TypeOptions UpperSaturationLimit: Saturation/Enabled/Saturation/UpperLimit | Saturation Fdbk/Enabled/Saturation/UpperLimit
      mask TypeOptions LowerSaturationLimit: Saturation/Enabled/Saturation/LowerLimit | Saturation Fdbk/Enabled/Saturation/LowerLimit
      mask TypeOptions LinearizeAsGain: Saturation/Enabled/Saturation/LinearizeAsGain | Saturation Fdbk/Enabled/Saturation/LinearizeAsGain | Anti-windup/Cont. Clamping Ideal/Dead Zone/Enabled/DeadZone/LinearizeAsGain | Anti-windup/Back Calculation/Kb/LinearizeAsGain | Anti-windup/Cont. Clamping Ideal/ZeroGain/LinearizeAsGain | Anti-windup/Cont. Clamping Parallel/Dead Zone/Enabled/DeadZone/LinearizeAsGain | Anti-windup/Cont. Clamping Parallel/ZeroGain/LinearizeAsGain | Anti-windup/Disc. Clamping Ideal/Dead Zone/Enabled/DeadZone/LinearizeAsGain | Anti-windup/Disc. Clamping Ideal/ZeroGain/LinearizeAsGain | Anti-windup/Disc. Clamping Parallel/Dead Zone/Enabled/DeadZone/LinearizeAsGain | Anti-windup/Disc. Clamping Parallel/ZeroGain/LinearizeAsGain | D Gain/Internal Parameters/Derivative Gain/LinearizeAsGain | Filter/Disc. Trapezoidal Filter/Tsamp/External Ts/Gain/LinearizeAsGain | I Gain/Internal Parameters/Integral Gain/LinearizeAsGain | Ideal P Gain/Internal Parameters/Proportional Gain/LinearizeAsGain | Ideal P Gain Fdbk/Internal Parameters/Proportional Gain/LinearizeAsGain | N Gain/Internal Parameters/Filter Coefficient/LinearizeAsGain | Parallel P Gain/Internal Parameters/Proportional Gain/LinearizeAsGain | Tracking Mode/Enabled/Kt/LinearizeAsGain
      mask TypeOptions AntiWindupMode: Simulink:masks:none | Simulink:masks:backCalculation | Simulink:masks:clamping | Simulink:masks:external
      mask Callback AntiWindupMode: pidpack.PIDConfig.callbackMaskVisibilities(gcbh)
      mask TypeOptions Kb: Anti-windup/Back Calculation/Kb/Gain
      mask TypeOptions LimitIntegrator: Integrator/Continuous/Integrator/LimitOutput | Integrator/Discrete/Integrator/LimitOutput
      mask Callback LimitIntegrator: pidpack.PIDConfig.callbackMaskVisibilities(gcbh)
      mask TypeOptions RndMeth:
      | Integrator/Discrete/Integrator/RndMeth | Anti-windup/Back Calculation/Kb/RndMeth | Anti-windup/Back Calculation/SumI4/RndMeth | Anti-windup/Back Calculation/SumI2/RndMeth | Anti-windup/Cont. Clamping Ideal/DataTypeConv1/RndMeth | Anti-windup/Cont. Clamping Ideal/DataTypeConv2/RndMeth | Anti-windup/Cont. Clamping Ideal/DataTypeConv4/RndMeth | Anti-windup/Cont. Clamping Ideal/Equal1/RndMeth | Anti-windup/Cont. Clamping Ideal/Equal2/RndMeth | Anti-windup/Cont. Clamping Ideal/NotEqual/RndMeth | Anti-windup/Cont. Clamping Ideal/Switch/RndMeth | Anti-windup/Cont. Clamping Ideal/ZeroGain/RndMeth | Anti-windup/Disc. Clamping Parallel/DataTypeConv1/RndMeth | Anti-windup/Disc. Clamping Parallel/DataTypeConv2/RndMeth | Anti-windup/Disc. Clamping Parallel/Equal1/RndMeth | Anti-windup/Disc. Clamping Parallel/NotEqual/RndMeth | Anti-windup/Disc. Clamping Parallel/Switch/RndMeth | Anti-windup/Disc. Clamping Parallel/ZeroGain/RndMeth | D Gain/External Parameters/DProd Out/RndMeth | D Gain/Internal Parameters/Derivative Gain/RndMeth | Filter/Cont. Filter/SumD/RndMeth | Filter/Differentiator/Diff/RndMeth | Filter/Disc. Backward Euler Filter/DenCoefOut/RndMeth | Filter/Disc. Backward Euler Filter/Filter Differentiator TF/RndMeth | Filter/Disc. Backward Euler Filter/Passthrough for tuning/RndMeth | Filter/Disc. Backward Euler Filter/Reciprocal/RndMeth | Filter/Disc. Backward Euler Filter/SumDen/RndMeth | Filter/Disc. Forward Euler Filter/Filter/RndMeth | Filter/Disc. Forward Euler Filter/SumD/RndMeth | Filter/Disc. Trapezoidal Filter/DenCoefOut/RndMeth | Filter/Disc. Trapezoidal Filter/Divide/RndMeth | Filter/Disc. Trapezoidal Filter/Filter Differentiator TF/RndMeth | Filter/Disc. Trapezoidal Filter/Passthrough for tuning/RndMeth | Filter/Disc. Trapezoidal Filter/Reciprocal/RndMeth | Filter/Disc. Trapezoidal Filter/SumDen/RndMeth | Filter/Disc. Trapezoidal Filter/SumNum/RndMeth | I Gain/External Parameters/IProd Out/RndMeth | I Gain/Internal Parameters/Integral Gain/RndMeth | Ideal P Gain/External Parameters/PProd Out/RndMeth | Ideal P Gain/Internal Parameters/Proportional Gain/RndMeth | Ideal P Gain Fdbk/External Parameters/PProd Out/RndMeth | Ideal P Gain Fdbk/Internal Parameters/Proportional Gain/RndMeth | N Gain/External Parameters/NProd Out/RndMeth | N Gain/Internal Parameters/Filter Coefficient/RndMeth | Parallel P Gain/External Parameters/PProd Out/RndMeth | Parallel P Gain/Internal Parameters/Proportional Gain/RndMeth | Saturation/Enabled/Saturation/RndMeth | Saturation Fdbk/Enabled/Saturation/RndMeth | Tracking Mode/Enabled/Kt/RndMeth | Tracking Mode/Enabled/SumI3/RndMeth | Anti-windup/Cont. Clamping Parallel/DataTypeConv1/RndMeth | Anti-windup/Cont. Clamping Parallel/DataTypeConv2/RndMeth | Anti-windup/Cont. Clamping Parallel/Equal1/RndMeth | Anti-windup/Cont. Clamping Parallel/NotEqual/RndMeth | Anti-windup/Cont. Clamping Parallel/Switch/RndMeth | Anti-windup/Cont. Clamping Parallel/ZeroGain/RndMeth | Anti-windup/Disc. Clamping Ideal/DataTypeConv1/RndMeth | Anti-windup/Disc. Clamping Ideal/DataTypeConv2/RndMeth | Anti-windup/Disc. Clamping Ideal/DataTypeConv4/RndMeth | Anti-windup/Disc. Clamping Ideal/Equal1/RndMeth | Anti-windup/Disc. Clamping Ideal/Equal2/RndMeth | Anti-windup/Disc. Clamping Ideal/NotEqual/RndMeth | Anti-windup/Disc. Clamping Ideal/Switch/RndMeth | Anti-windup/Disc. Clamping Ideal/ZeroGain/RndMeth | Sum/Sum_PD/Sum/RndMeth | Sum/Sum_PI/Sum/RndMeth | Sum/Sum_PID/Sum/RndMeth | Sum Fdbk/Enabled/Sum Fdbk/RndMeth | Tracking Mode Sum/Tracking Mode/SumI1/RndMeth | Filter/Differentiator/Tsamp/External Ts/Udiff*Ts Prod Out/RndMeth | Filter/Differentiator/Tsamp/Internal Ts/Tsamp/RndMeth | Filter/Disc. Backward Euler Filter/Tsamp/External Ts/N*Ts Prod Out/RndMeth | Filter/Disc. Backward Euler Filter/Tsamp/Internal Ts/Tsamp/RndMeth | Filter/Disc. Trapezoidal Filter/Tsamp/External Ts/N*Ts Prod Out/RndMeth | Filter/Disc. Trapezoidal Filter/Tsamp/Internal Ts/Tsamp/RndMeth | Tsamp - Integral/External Ts/Uintegral*Ts Prod Out/RndMeth | Tsamp - Ngain/External Ts/Ungain*Ts Prod Out/RndMeth | Filter/Disc. Trapezoidal Filter/Tsamp/External Ts/Gain/RndMeth | Saturation/External/Saturation
      | Dynamic/RndMeth | Saturation Fdbk/External/Saturation
      | Dynamic/RndMeth
      mask TypeOptions SaturateOnIntegerOverflow:
      | Integrator/Discrete/Integrator/SaturateOnIntegerOverflow | Anti-windup/Back Calculation/Kb/SaturateOnIntegerOverflow | Anti-windup/Back Calculation/SumI4/SaturateOnIntegerOverflow | Anti-windup/Back Calculation/SumI2/SaturateOnIntegerOverflow | Anti-windup/Cont. Clamping Ideal/DataTypeConv1/SaturateOnIntegerOverflow | Anti-windup/Cont. Clamping Ideal/DataTypeConv2/SaturateOnIntegerOverflow | Anti-windup/Cont. Clamping Ideal/DataTypeConv4/SaturateOnIntegerOverflow | Anti-windup/Cont. Clamping Ideal/Switch/SaturateOnIntegerOverflow | Anti-windup/Cont. Clamping Ideal/ZeroGain/SaturateOnIntegerOverflow | Anti-windup/Disc. Clamping Parallel/DataTypeConv1/SaturateOnIntegerOverflow | Anti-windup/Disc. Clamping Parallel/DataTypeConv2/SaturateOnIntegerOverflow | Anti-windup/Disc. Clamping Parallel/Switch/SaturateOnIntegerOverflow | Anti-windup/Disc. Clamping Parallel/ZeroGain/SaturateOnIntegerOverflow | D Gain/External Parameters/DProd Out/SaturateOnIntegerOverflow | D Gain/Internal Parameters/Derivative Gain/SaturateOnIntegerOverflow | Filter/Cont. Filter/SumD/SaturateOnIntegerOverflow | Filter/Differentiator/Diff/SaturateOnIntegerOverflow | Filter/Disc. Backward Euler Filter/DenCoefOut/SaturateOnIntegerOverflow | Filter/Disc. Backward Euler Filter/Filter Differentiator TF/SaturateOnIntegerOverflow | Filter/Disc. Backward Euler Filter/Passthrough for tuning/SaturateOnIntegerOverflow | Filter/Disc. Backward Euler Filter/Reciprocal/SaturateOnIntegerOverflow | Filter/Disc. Backward Euler Filter/SumDen/SaturateOnIntegerOverflow | Filter/Disc. Backward Euler Filter/Unary Minus/SaturateOnIntegerOverflow | Filter/Disc. Forward Euler Filter/Filter/SaturateOnIntegerOverflow | Filter/Disc. Forward Euler Filter/SumD/SaturateOnIntegerOverflow | Filter/Disc. Trapezoidal Filter/DenCoefOut/SaturateOnIntegerOverflow | Filter/Disc. Trapezoidal Filter/Divide/SaturateOnIntegerOverflow | Filter/Disc. Trapezoidal Filter/Filter Differentiator TF/SaturateOnIntegerOverflow | Filter/Disc. Trapezoidal Filter/Passthrough for tuning/SaturateOnIntegerOverflow | Filter/Disc. Trapezoidal Filter/Reciprocal/SaturateOnIntegerOverflow | Filter/Disc. Trapezoidal Filter/SumDen/SaturateOnIntegerOverflow | Filter/Disc. Trapezoidal Filter/SumNum/SaturateOnIntegerOverflow | I Gain/External Parameters/IProd Out/SaturateOnIntegerOverflow | I Gain/Internal Parameters/Integral Gain/SaturateOnIntegerOverflow | Ideal P Gain/External Parameters/PProd Out/SaturateOnIntegerOverflow | Ideal P Gain/Internal Parameters/Proportional Gain/SaturateOnIntegerOverflow | Ideal P Gain Fdbk/External Parameters/PProd Out/SaturateOnIntegerOverflow | Ideal P Gain Fdbk/Internal Parameters/Proportional Gain/SaturateOnIntegerOverflow | N Gain/External Parameters/NProd Out/SaturateOnIntegerOverflow | N Gain/Internal Parameters/Filter Coefficient/SaturateOnIntegerOverflow | Parallel P Gain/External Parameters/PProd Out/SaturateOnIntegerOverflow | Parallel P Gain/Internal Parameters/Proportional Gain/SaturateOnIntegerOverflow | Tracking Mode/Enabled/Kt/SaturateOnIntegerOverflow | Tracking Mode/Enabled/SumI3/SaturateOnIntegerOverflow | Anti-windup/Cont. Clamping Parallel/DataTypeConv1/SaturateOnIntegerOverflow | Anti-windup/Cont. Clamping Parallel/DataTypeConv2/SaturateOnIntegerOverflow | Anti-windup/Cont. Clamping Parallel/Switch/SaturateOnIntegerOverflow | Anti-windup/Cont. Clamping Parallel/ZeroGain/SaturateOnIntegerOverflow | Anti-windup/Disc. Clamping Ideal/DataTypeConv1/SaturateOnIntegerOverflow | Anti-windup/Disc. Clamping Ideal/DataTypeConv2/SaturateOnIntegerOverflow | Anti-windup/Disc. Clamping Ideal/DataTypeConv4/SaturateOnIntegerOverflow | Anti-windup/Disc. Clamping Ideal/Switch/SaturateOnIntegerOverflow | Anti-windup/Disc. Clamping Ideal/ZeroGain/SaturateOnIntegerOverflow | Sum/Sum_PD/Sum/SaturateOnIntegerOverflow | Sum/Sum_PI/Sum/SaturateOnIntegerOverflow | Sum/Sum_PID/Sum/SaturateOnIntegerOverflow | Sum Fdbk/Enabled/Sum Fdbk/SaturateOnIntegerOverflow | Tracking Mode Sum/Tracking Mode/SumI1/SaturateOnIntegerOverflow | Filter/Differentiator/Tsamp/External Ts/Udiff*Ts Prod Out/SaturateOnIntegerOverflow | Filter/Differentiator/Tsamp/Internal Ts/Tsamp/SaturateOnIntegerOverflow | Filter/Disc. Backward Euler Filter/Tsamp/External Ts/N*Ts Prod Out/SaturateOnIntegerOverflow | Filter/Disc. Backward Euler Filter/Tsamp/Internal Ts/Tsamp/SaturateOnIntegerOverflow | Filter/Disc. Trapezoidal Filter/Tsamp/External Ts/N*Ts Prod Out/SaturateOnIntegerOverflow | Filter/Disc. Trapezoidal Filter/Tsamp/Internal Ts/Tsamp/SaturateOnIntegerOverflow | Tsamp - Integral/External Ts/Uintegral*Ts Prod Out/SaturateOnIntegerOverflow | Tsamp - Ngain/External Ts/Ungain*Ts Prod Out/SaturateOnIntegerOverflow | Filter/Disc. Trapezoidal Filter/Tsamp/External Ts/Gain/SaturateOnIntegerOverflow | Saturation/External/Saturation
      | Dynamic/DoSatur | Saturation Fdbk/External/Saturation
      | Dynamic/DoSatur | Anti-windup/Cont. Clamping Ideal/Dead Zone/Enabled/DeadZone/SaturateOnIntegerOverflow | Anti-windup/Cont. Clamping Parallel/Dead Zone/Enabled/DeadZone/SaturateOnIntegerOverflow | Anti-windup/Disc. Clamping Ideal/Dead Zone/Enabled/DeadZone/SaturateOnIntegerOverflow | Anti-windup/Disc. Clamping Parallel/Dead Zone/Enabled/DeadZone/SaturateOnIntegerOverflow
      mask TypeOptions LockScale: Integrator/Discrete/Integrator/LockScale | Anti-windup/preSat/LockScale | Anti-windup/postSat/LockScale | Anti-windup/P/LockScale | Anti-windup/preInt/LockScale | Anti-windup/Back Calculation/preSat/LockScale | Anti-windup/Back Calculation/postSat/LockScale | Anti-windup/Back Calculation/preInt/LockScale | Anti-windup/Back Calculation/Kb/LockScale | Anti-windup/Back Calculation/SumI4/LockScale | Anti-windup/Back Calculation/SumI2/LockScale | Anti-windup/Back Calculation/Out1/LockScale | Anti-windup/Cont. Clamping Ideal/preSat/LockScale | Anti-windup/Cont. Clamping Ideal/P/LockScale | Anti-windup/Cont. Clamping Ideal/preInt/LockScale | Anti-windup/Cont. Clamping Ideal/Constant/LockScale | Anti-windup/Cont. Clamping Ideal/Constant1/LockScale | Anti-windup/Cont. Clamping Ideal/DataTypeConv1/LockScale | Anti-windup/Cont. Clamping Ideal/DataTypeConv2/LockScale | Anti-windup/Cont. Clamping Ideal/DataTypeConv4/LockScale | Anti-windup/Cont. Clamping Ideal/Switch/LockScale | Anti-windup/Cont. Clamping Ideal/ZeroGain/LockScale | Anti-windup/Cont. Clamping Ideal/Out1/LockScale | Anti-windup/Disc. Clamping Parallel/preSat/LockScale | Anti-windup/Disc. Clamping Parallel/preInt/LockScale | Anti-windup/Disc. Clamping Parallel/Constant1/LockScale | Anti-windup/Disc. Clamping Parallel/DataTypeConv1/LockScale | Anti-windup/Disc. Clamping Parallel/DataTypeConv2/LockScale | Anti-windup/Disc. Clamping Parallel/Switch/LockScale | Anti-windup/Disc. Clamping Parallel/ZeroGain/LockScale | Anti-windup/Disc. Clamping Parallel/Out1/LockScale | Anti-windup/Passthrough/Out1/LockScale | Anti-windup/Out1/LockScale | D Gain/err/LockScale | D Gain/D Gain/LockScale | D Gain/External Parameters/err/LockScale | D Gain/External Parameters/D Gain/LockScale | D Gain/External Parameters/DProd Out/LockScale | D Gain/External Parameters/Out1/LockScale | D Gain/Internal Parameters/err/LockScale | D Gain/Internal Parameters/Derivative Gain/LockScale | D Gain/Internal Parameters/Out1/LockScale | D Gain/Out1/LockScale | Filter/Reset/LockScale | Filter/U/LockScale | Filter/N/LockScale | Filter/D0in/LockScale | Filter/Nout/LockScale | Filter/Cont. Filter/U/LockScale | Filter/Cont. Filter/Nout/LockScale | Filter/Cont. Filter/Reset/LockScale | Filter/Cont. Filter/D0in/LockScale | Filter/Cont. Filter/SumD/LockScale | Filter/Cont. Filter/Y/LockScale | Filter/Differentiator/U/LockScale | Filter/Differentiator/Reset/LockScale | Filter/Differentiator/D0in/LockScale | Filter/Differentiator/Diff/LockScale | Filter/Differentiator/Y/LockScale | Filter/Disc. Backward Euler Filter/U/LockScale | Filter/Disc. Backward Euler Filter/N/LockScale | Filter/Disc. Backward Euler Filter/Reset/LockScale | Filter/Disc. Backward Euler Filter/D0in/LockScale | Filter/Disc. Backward Euler Filter/Constant/LockScale | Filter/Disc. Backward Euler Filter/DenCoefOut/LockScale | Filter/Disc. Backward Euler Filter/Filter Differentiator TF/LockScale | Filter/Disc. Backward Euler Filter/Passthrough for tuning/LockScale | Filter/Disc. Backward Euler Filter/Reciprocal/LockScale | Filter/Disc. Backward Euler Filter/SumDen/LockScale | Filter/Disc. Backward Euler Filter/Y/LockScale | Filter/Disc. Forward Euler Filter/U/LockScale | Filter/Disc. Forward Euler Filter/Nout/LockScale | Filter/Disc. Forward Euler Filter/Reset/LockScale | Filter/Disc. Forward Euler Filter/D0in/LockScale | Filter/Disc. Forward Euler Filter/Filter/LockScale | Filter/Disc. Forward Euler Filter/SumD/LockScale | Filter/Disc. Forward Euler Filter/Y/LockScale | Filter/Disc. Trapezoidal Filter/U/LockScale | Filter/Disc. Trapezoidal Filter/N/LockScale | Filter/Disc. Trapezoidal Filter/Reset/LockScale | Filter/Disc. Trapezoidal Filter/D0in/LockScale | Filter/Disc. Trapezoidal Filter/Constant/LockScale | Filter/Disc. Trapezoidal Filter/DenCoefOut/LockScale | Filter/Disc. Trapezoidal Filter/Divide/LockScale | Filter/Disc. Trapezoidal Filter/Filter Differentiator TF/LockScale | Filter/Disc. Trapezoidal Filter/Passthrough for tuning/LockScale | Filter/Disc. Trapezoidal Filter/Reciprocal/LockScale | Filter/Disc. Trapezoidal Filter/SumDen/LockScale | Filter/Disc. Trapezoidal Filter/SumNum/LockScale | Filter/Disc. Trapezoidal Filter/Y/LockScale | Filter/Y/LockScale | Filter ICs/D0/LockScale | Filter ICs/External IC/D0/LockScale | Filter ICs/External IC/Out1/LockScale | Filter ICs/Internal IC - Differentiator/Out1/LockScale | Filter ICs/Internal IC - Filter/Out1/LockScale | Filter ICs/Out1/LockScale | I Gain/err/LockScale | I Gain/I Gain/LockScale | I Gain/External Parameters/err/LockScale | I Gain/External Parameters/I Gain/LockScale | I Gain/External Parameters/IProd Out/LockScale | I Gain/External Parameters/Out1/LockScale | I Gain/Internal Parameters/err/LockScale | I Gain/Internal Parameters/Integral Gain/LockScale | I Gain/Internal Parameters/Out1/LockScale | I Gain/Out1/LockScale | Ideal P Gain/In1/LockScale | Ideal P Gain/P Gain/LockScale | Ideal P Gain/External Parameters/In1/LockScale | Ideal P Gain/External Parameters/P Gain/LockScale | Ideal P Gain/External Parameters/PProd Out/LockScale | Ideal P Gain/External Parameters/Out1/LockScale | Ideal P Gain/Internal Parameters/In1/LockScale | Ideal P Gain/Internal Parameters/Proportional Gain/LockScale | Ideal P Gain/Internal Parameters/Out1/LockScale | Ideal P Gain/Passthrough/In1/LockScale | Ideal P Gain/Passthrough/Out1/LockScale | Ideal P Gain/Out1/LockScale | Ideal P Gain Fdbk/In1/LockScale | Ideal P Gain Fdbk/P Gain/LockScale | Ideal P Gain Fdbk/External Parameters/In1/LockScale | Ideal P Gain Fdbk/External Parameters/P Gain/LockScale | Ideal P Gain Fdbk/External Parameters/PProd Out/LockScale | Ideal P Gain Fdbk/External Parameters/Out1/LockScale | Ideal P Gain Fdbk/Internal Parameters/In1/LockScale | Ideal P Gain Fdbk/Internal Parameters/Proportional Gain/LockScale | Ideal P Gain Fdbk/Internal Parameters/Out1/LockScale | Ideal P Gain Fdbk/Passthrough/In1/LockScale | Ideal P Gain Fdbk/Passthrough/Out1/LockScale | Ideal P Gain Fdbk/Out1/LockScale | Integrator/U/LockScale | Integrator/I0in/LockScale | Integrator/Reset/LockScale | Integrator/Continuous/U/LockScale | Integrator/Continuous/Reset/LockScale | Integrator/Continuous/I0in/LockScale | Integrator/Continuous/out/LockScale | Integrator/Discrete/U/LockScale | Integrator/Discrete/Reset/LockScale | Integrator/Discrete/I0in/LockScale | Integrator/Discrete/out/LockScale | Integrator/Discrete/state/LockScale | Integrator/state/LockScale | Integrator/out/LockScale | Integrator ICs/I0/LockScale | Integrator ICs/External IC/I0/LockScale | Integrator ICs/External IC/Out1/LockScale | Integrator ICs/Internal IC/Out1/LockScale | Integrator ICs/Out1/LockScale | N Copy/N Gain/LockScale | N Copy/External Parameters/N Gain/LockScale | N Copy/External Parameters/Out1/LockScale | N Copy/Internal Parameters/N Copy/LockScale | N Copy/Internal Parameters/Out1/LockScale | N Copy/Out1/LockScale | N Gain/U/LockScale | N Gain/N Gain/LockScale | N Gain/External Parameters/U/LockScale | N Gain/External Parameters/N Gain/LockScale | N Gain/External Parameters/NProd Out/LockScale | N Gain/External Parameters/Out1/LockScale | N Gain/Internal Parameters/U/LockScale | N Gain/Internal Parameters/Filter Coefficient/LockScale | N Gain/Internal Parameters/Out1/LockScale | N Gain/Passthrough/U/LockScale | N Gain/Passthrough/Out1/LockScale | N Gain/Out1/LockScale | P Copy/P Gain/LockScale | P Copy/External Parameters Ideal/P Gain/LockScale | P Copy/External Parameters Ideal/Out1/LockScale | P Copy/Internal Parameters Ideal/P Copy/LockScale | P Copy/Internal Parameters Ideal/Out1/LockScale | P Copy/Out1/LockScale | Parallel P Gain/err/LockScale | Parallel P Gain/P Gain/LockScale | Parallel P Gain/External Parameters/err/LockScale | Parallel P Gain/External Parameters/P Gain/LockScale | Parallel P Gain/External Parameters/PProd Out/LockScale | Parallel P Gain/External Parameters/Out1/LockScale | Parallel P Gain/Internal Parameters/err/LockScale | Parallel P Gain/Internal Parameters/Proportional Gain/LockScale | Parallel P Gain/Internal Parameters/Out1/LockScale | Parallel P Gain/Passthrough/err/LockScale | Parallel P Gain/Passthrough/Out1/LockScale | Parallel P Gain/Out1/LockScale | Saturation/In1/LockScale | Saturation/Enabled/In1/LockScale | Saturation/Enabled/Saturation/LockScale | Saturation/Enabled/Out1/LockScale | Saturation/Passthrough/In1/LockScale | Saturation/Passthrough/Out1/LockScale | Saturation/Out1/LockScale | Saturation Fdbk/In1/LockScale | Saturation Fdbk/Enabled/In1/LockScale | Saturation Fdbk/Enabled/Saturation/LockScale | Saturation Fdbk/Enabled/Out1/LockScale | Saturation Fdbk/Passthrough/In1/LockScale | Saturation Fdbk/Passthrough/Out1/LockScale | Saturation Fdbk/Out1/LockScale | Tracking Mode/uout/LockScale | Tracking Mode/TR/LockScale | Tracking Mode/Enabled/uout/LockScale | Tracking Mode/Enabled/TR/LockScale | Tracking Mode/Enabled/Kt/LockScale | Tracking Mode/Enabled/SumI3/LockScale | Tracking Mode/Enabled/Out1/LockScale | Tracking Mode/Out1/LockScale | postSat Signal/feedback/LockScale | postSat Signal/forward/LockScale | postSat Signal/Feedback_Path/feedback/LockScale | postSat Signal/Feedback_Path/Out1/LockScale | postSat Signal/Forward_Path/forward/LockScale | postSat Signal/Forward_Path/Out1/LockScale | postSat Signal/Out1/LockScale | preSat Signal/feedback/LockScale | preSat Signal/forward/LockScale | preSat Signal/Feedback_Path/feedback/LockScale | preSat Signal/Feedback_Path/Out1/LockScale | preSat Signal/Forward_Path/forward/LockScale | preSat Signal/Forward_Path/Out1/LockScale | preSat Signal/Out1/LockScale | Anti-windup/Cont. Clamping Parallel/preSat/LockScale | Anti-windup/Cont. Clamping Parallel/preInt/LockScale | Anti-windup/Cont. Clamping Parallel/Constant1/LockScale | Anti-windup/Cont. Clamping Parallel/DataTypeConv1/LockScale | Anti-windup/Cont. Clamping Parallel/DataTypeConv2/LockScale | Anti-windup/Cont. Clamping Parallel/Switch/LockScale | Anti-windup/Cont. Clamping Parallel/ZeroGain/LockScale | Anti-windup/Cont. Clamping Parallel/Out1/LockScale | Anti-windup/Disc. Clamping Ideal/preSat/LockScale | Anti-windup/Disc. Clamping Ideal/P/LockScale | Anti-windup/Disc. Clamping Ideal/preInt/LockScale | Anti-windup/Disc. Clamping Ideal/Constant/LockScale | Anti-windup/Disc. Clamping Ideal/Constant1/LockScale | Anti-windup/Disc. Clamping Ideal/DataTypeConv1/LockScale | Anti-windup/Disc. Clamping Ideal/DataTypeConv2/LockScale | Anti-windup/Disc. Clamping Ideal/DataTypeConv4/LockScale | Anti-windup/Disc. Clamping Ideal/Switch/LockScale | Anti-windup/Disc. Clamping Ideal/ZeroGain/LockScale | Anti-windup/Disc. Clamping Ideal/Out1/LockScale | Reset Signal/Reset/LockScale | Reset Signal/External Reset/Reset/LockScale | Reset Signal/External Reset/Out1/LockScale | Reset Signal/Out1/LockScale | Anti-windup/Back Calculation/P/LockScale | Anti-windup/Back Calculation/Signal Specification2/LockScale | Anti-windup/Cont. Clamping Ideal/postSat/LockScale | Anti-windup/Cont. Clamping Parallel/postSat/LockScale | Anti-windup/Cont. Clamping Parallel/P/LockScale | Anti-windup/Cont. Clamping Parallel/Signal Specification2/LockScale | Anti-windup/Disabled/preInt/LockScale | Anti-windup/Disabled/preSat/LockScale | Anti-windup/Disabled/postSat/LockScale | Anti-windup/Disabled/P/LockScale | Anti-windup/Disabled/Signal Specification1/LockScale | Anti-windup/Disabled/Signal Specification2/LockScale | Anti-windup/Disc. Clamping Ideal/postSat/LockScale | Anti-windup/Disc. Clamping Parallel/postSat/LockScale | Anti-windup/Disc. Clamping Parallel/P/LockScale | Anti-windup/Disc. Clamping Parallel/Signal Specification2/LockScale | Anti-windup/Passthrough/preInt/LockScale | Anti-windup/Passthrough/preSat/LockScale | Anti-windup/Passthrough/postSat/LockScale | Anti-windup/Passthrough/P/LockScale | Anti-windup/Passthrough/Signal Specification2/LockScale | D Gain/Disabled/D Gain/LockScale | D Gain/Disabled/Signal Specification/LockScale | D Gain/Internal Parameters/D Gain/LockScale | D Gain/Internal Parameters/Signal Specification/LockScale | Filter/Cont. Filter/N/LockScale | Filter/Cont. Filter/Signal Specification2/LockScale | Filter/Differentiator/Nout/LockScale | Filter/Differentiator/N/LockScale | Filter/Differentiator/Signal Specification1/LockScale | Filter/Disabled/Reset/LockScale | Filter/Disabled/U/LockScale | Filter/Disabled/N/LockScale | Filter/Disabled/D0in/LockScale | Filter/Disabled/Nout/LockScale | Filter/Disabled/Signal Specification1/LockScale | Filter/Disabled/Signal Specification2/LockScale | Filter/Disabled/Signal Specification3/LockScale | Filter/Disabled/Signal Specification4/LockScale | Filter/Disc. Backward Euler Filter/Nout/LockScale | Filter/Disc. Forward Euler Filter/N/LockScale | Filter/Disc. Forward Euler Filter/Signal Specification2/LockScale | Filter/Disc. Trapezoidal Filter/Nout/LockScale | Filter ICs/Disabled/D0/LockScale | Filter ICs/Disabled/Signal Specification/LockScale | Filter ICs/Disabled/Signal Specification1/LockScale | Filter ICs/Disabled/Out1/LockScale | Filter ICs/Internal IC - Differentiator/D0/LockScale | Filter ICs/Internal IC - Differentiator/Signal Specification/LockScale | Filter ICs/Internal IC - Differentiator/Signal Specification1/LockScale | Filter ICs/Internal IC - Filter/D0/LockScale | Filter ICs/Internal IC - Filter/Signal Specification/LockScale | Filter ICs/Internal IC - Filter/Signal Specification1/LockScale | I Gain/Disabled/I Gain/LockScale | I Gain/Disabled/Signal Specification/LockScale | I Gain/Internal Parameters/I Gain/LockScale | I Gain/Internal Parameters/Signal Specification/LockScale | Ideal P Gain/Internal Parameters/P Gain/LockScale | Ideal P Gain/Internal Parameters/Signal Specification1/LockScale | Ideal P Gain/Passthrough/P Gain/LockScale | Ideal P Gain Fdbk/Disabled/In1/LockScale | Ideal P Gain Fdbk/Disabled/P Gain/LockScale | Ideal P Gain Fdbk/Disabled/Signal Specification1/LockScale | Ideal P Gain Fdbk/Internal Parameters/P Gain/LockScale | Ideal P Gain Fdbk/Internal Parameters/Signal Specification1/LockScale | Ideal P Gain Fdbk/Passthrough/P Gain/LockScale | Integrator/Continuous/Signal Specification1/LockScale | Integrator/Continuous/state/LockScale | Integrator/Disabled/U/LockScale | Integrator/Disabled/Reset/LockScale | Integrator/Disabled/I0in/LockScale | Integrator/Disabled/Signal Specification1/LockScale | Integrator/Disabled/Signal Specification2/LockScale | Integrator/Disabled/Signal Specification4/LockScale | Integrator/Disabled/out/LockScale | Integrator/Discrete/Signal Specification1/LockScale | Integrator ICs/Disabled/I0/LockScale | Integrator ICs/Disabled/Signal Specification/LockScale | Integrator ICs/Disabled/Signal Specification1/LockScale | Integrator ICs/Disabled/Out1/LockScale | Integrator ICs/Internal IC/I0/LockScale | Integrator ICs/Internal IC/Signal Specification/LockScale | Integrator ICs/Internal IC/Signal Specification1/LockScale | N Copy/Disabled/N Gain/LockScale | N Copy/Disabled wSignal Specification/N Gain/LockScale | N Copy/Disabled wSignal Specification/Signal Specification1/LockScale | N Copy/Internal Parameters/N Gain/LockScale | N Copy/Internal Parameters/Signal Specification/LockScale | N Gain/Disabled/U/LockScale | N Gain/Disabled/N Gain/LockScale | N Gain/Disabled/Signal Specification1/LockScale | N Gain/Disabled/Signal Specification2/LockScale | N Gain/Internal Parameters/N Gain/LockScale | N Gain/Internal Parameters/Signal Specification1/LockScale | N Gain/Passthrough/N Gain/LockScale | P Copy/Disabled/P Gain/LockScale | P Copy/Internal Parameters Ideal/P Gain/LockScale | Parallel P Gain/Disabled/P Gain/LockScale | Parallel P Gain/Disabled/Signal Specification/LockScale | Parallel P Gain/Internal Parameters/P Gain/LockScale | Parallel P Gain/Internal Parameters/Signal Specification/LockScale | Parallel P Gain/Passthrough/P Gain/LockScale | Reset Signal/Disabled/Reset/LockScale | Reset Signal/Disabled/Signal Specification/LockScale | Reset Signal/Disabled/Signal Specification1/LockScale | Reset Signal/Disabled/Out1/LockScale | Saturation Fdbk/Disabled/In1/LockScale | Saturation Fdbk/Disabled/Signal Specification1/LockScale | Sum/P/LockScale | Sum/I/LockScale | Sum/D/LockScale | Sum/Passthrough_I/I/LockScale | Sum/Passthrough_I/Out1/LockScale | Sum/Passthrough_P/P/LockScale | Sum/Passthrough_P/Out1/LockScale | Sum/Sum_PD/P/LockScale | Sum/Sum_PD/D/LockScale | Sum/Sum_PD/Sum/LockScale | Sum/Sum_PD/Out1/LockScale | Sum/Sum_PI/P/LockScale | Sum/Sum_PI/I/LockScale | Sum/Sum_PI/Sum/LockScale | Sum/Sum_PI/Out1/LockScale | Sum/Sum_PID/P/LockScale | Sum/Sum_PID/I/LockScale | Sum/Sum_PID/D/LockScale | Sum/Sum_PID/Sum/LockScale | Sum/Sum_PID/Out1/LockScale | Sum/Out1/LockScale | Sum Fdbk/fromP/LockScale | Sum Fdbk/fromState/LockScale | Sum Fdbk/fromD/LockScale | Sum Fdbk/Disabled/fromP/LockScale | Sum Fdbk/Disabled/fromState/LockScale | Sum Fdbk/Disabled/fromD/LockScale | Sum Fdbk/Disabled/Signal Specification1/LockScale | Sum Fdbk/Enabled/fromP/LockScale | Sum Fdbk/Enabled/fromState/LockScale | Sum Fdbk/Enabled/fromD/LockScale | Sum Fdbk/Enabled/Sum Fdbk/LockScale | Sum Fdbk/Enabled/Out1/LockScale | Sum Fdbk/Passthrough/fromState/LockScale | Sum Fdbk/Passthrough/Out1/LockScale | Sum Fdbk/Out1/LockScale | Tracking Mode/Disabled/uout/LockScale | Tracking Mode/Disabled/TR/LockScale | Tracking Mode/Disabled/Signal Specification1/LockScale | Tracking Mode Sum/fromIgain/LockScale | Tracking Mode Sum/fromTR/LockScale | Tracking Mode Sum/Passthrough/fromIgain/LockScale | Tracking Mode Sum/Passthrough/fromTR/LockScale | Tracking Mode Sum/Passthrough/Signal Specification/LockScale | Tracking Mode Sum/Passthrough/Out1/LockScale | Tracking Mode Sum/Tracking Mode/fromIgain/LockScale | Tracking Mode Sum/Tracking Mode/fromTR/LockScale | Tracking Mode Sum/Tracking Mode/SumI1/LockScale | Tracking Mode Sum/Tracking Mode/Out1/LockScale | Tracking Mode Sum/Out1/LockScale | postSat Signal/Feedback_Path/forward/LockScale | postSat Signal/Forward_Path/feedback/LockScale | postSat Signal/Forward_Path/Signal Specification1/LockScale | preSat Signal/Feedback_Path/forward/LockScale | preSat Signal/Forward_Path/feedback/LockScale | preSat Signal/Forward_Path/Signal Specification1/LockScale | Filter/Ts/LockScale | Filter/Cont. Filter/Ts/LockScale | Filter/Differentiator/Ts/LockScale | Filter/Differentiator/Tsamp/U/LockScale | Filter/Differentiator/Tsamp/Ts/LockScale | Filter/Differentiator/Tsamp/External Ts/U/LockScale | Filter/Differentiator/Tsamp/External Ts/Ts/LockScale | Filter/Differentiator/Tsamp/External Ts/Udiff*Ts Prod Out/LockScale | Filter/Differentiator/Tsamp/External Ts/Out1/LockScale | Filter/Differentiator/Tsamp/Internal Ts/U/LockScale | Filter/Differentiator/Tsamp/Internal Ts/Ts/LockScale | Filter/Differentiator/Tsamp/Internal Ts/Out1/LockScale | Filter/Differentiator/Tsamp/Out1/LockScale | Filter/Disabled/Ts/LockScale | Filter/Disc. Backward Euler Filter/Ts/LockScale | Filter/Disc. Backward Euler Filter/Tsamp/N/LockScale | Filter/Disc. Backward Euler Filter/Tsamp/Ts/LockScale | Filter/Disc. Backward Euler Filter/Tsamp/External Ts/N/LockScale | Filter/Disc. Backward Euler Filter/Tsamp/External Ts/Ts/LockScale | Filter/Disc. Backward Euler Filter/Tsamp/External Ts/N*Ts Prod Out/LockScale | Filter/Disc. Backward Euler Filter/Tsamp/External Ts/Out1/LockScale | Filter/Disc. Backward Euler Filter/Tsamp/Internal Ts/N/LockScale | Filter/Disc. Backward Euler Filter/Tsamp/Internal Ts/Ts/LockScale | Filter/Disc. Backward Euler Filter/Tsamp/Internal Ts/Out1/LockScale | Filter/Disc. Backward Euler Filter/Tsamp/Out1/LockScale | Filter/Disc. Forward Euler Filter/Ts/LockScale | Filter/Disc. Trapezoidal Filter/Ts/LockScale | Filter/Disc. Trapezoidal Filter/Tsamp/N/LockScale | Filter/Disc. Trapezoidal Filter/Tsamp/Ts/LockScale | Filter/Disc. Trapezoidal Filter/Tsamp/External Ts/N/LockScale | Filter/Disc. Trapezoidal Filter/Tsamp/External Ts/Ts/LockScale | Filter/Disc. Trapezoidal Filter/Tsamp/External Ts/N*Ts Prod Out/LockScale | Filter/Disc. Trapezoidal Filter/Tsamp/External Ts/Out1/LockScale | Filter/Disc. Trapezoidal Filter/Tsamp/Internal Ts/N/LockScale | Filter/Disc. Trapezoidal Filter/Tsamp/Internal Ts/Ts/LockScale | Filter/Disc. Trapezoidal Filter/Tsamp/Internal Ts/Out1/LockScale | Filter/Disc. Trapezoidal Filter/Tsamp/Out1/LockScale | Tsamp - Integral/U/LockScale | Tsamp - Integral/Ts/LockScale | Tsamp - Integral/Disabled/U/LockScale | Tsamp - Integral/Disabled/Ts/LockScale | Tsamp - Integral/Disabled/Out1/LockScale | Tsamp - Integral/Disabled wSignal Specification/U/LockScale | Tsamp - Integral/Disabled wSignal Specification/Ts/LockScale | Tsamp - Integral/Disabled wSignal Specification/Signal Specification/LockScale | Tsamp - Integral/Disabled wSignal Specification/Out1/LockScale | Tsamp - Integral/External Ts/U/LockScale | Tsamp - Integral/External Ts/Ts/LockScale | Tsamp - Integral/External Ts/Uintegral*Ts Prod Out/LockScale | Tsamp - Integral/External Ts/Out1/LockScale | Tsamp - Integral/Passthrough/U/LockScale | Tsamp - Integral/Passthrough/Ts/LockScale | Tsamp - Integral/Passthrough/Signal Specification/LockScale | Tsamp - Integral/Passthrough/Out1/LockScale | Tsamp - Integral/Out1/LockScale | Tsamp - Ngain/U/LockScale | Tsamp - Ngain/Ts/LockScale | Tsamp - Ngain/External Ts/U/LockScale | Tsamp - Ngain/External Ts/Ts/LockScale | Tsamp - Ngain/External Ts/Ungain*Ts Prod Out/LockScale | Tsamp - Ngain/External Ts/Out1/LockScale | Tsamp - Ngain/Passthrough/U/LockScale | Tsamp - Ngain/Passthrough/Ts/LockScale | Tsamp - Ngain/Passthrough/Out1/LockScale | Tsamp - Ngain/Out1/LockScale | y/LockScale
      mask TypeOptions PGainOutDataTypeStr: Parallel P Gain/Internal Parameters/Proportional Gain/OutDataTypeStr | Ideal P Gain/Internal Parameters/Proportional Gain/OutDataTypeStr | Ideal P Gain Fdbk/Internal Parameters/Proportional Gain/OutDataTypeStr
      mask Callback PGainOutDataTypeStr: pidpack.PIDConfig.callbackSyncDataType(gcbh, 'PGainOutDataTypeStr')
      mask TypeOptions PProdOutDataTypeStr: Parallel P Gain/External Parameters/PProd Out/OutDataTypeStr | Ideal P Gain/External Parameters/PProd Out/OutDataTypeStr | Ideal P Gain Fdbk/External Parameters/PProd Out/OutDataTypeStr
      mask Callback PProdOutDataTypeStr: pidpack.PIDConfig.callbackSyncDataType(gcbh, 'PProdOutDataTypeStr')
      mask TypeOptions POutMin: Parallel P Gain/Internal Parameters/Proportional Gain/OutMin | Parallel P Gain/External Parameters/PProd Out/OutMin | Ideal P Gain/Internal Parameters/Proportional Gain/OutMin | Ideal P Gain Fdbk/Internal Parameters/Proportional Gain/OutMin
      mask TypeOptions POutMax: Parallel P Gain/Internal Parameters/Proportional Gain/OutMax | Parallel P Gain/External Parameters/PProd Out/OutMax | Ideal P Gain/Internal Parameters/Proportional Gain/OutMax | Ideal P Gain Fdbk/Internal Parameters/Proportional Gain/OutMax
      mask TypeOptions IGainOutDataTypeStr: I Gain/Internal Parameters/Integral Gain/OutDataTypeStr
      mask Callback IGainOutDataTypeStr: pidpack.PIDConfig.callbackSyncDataType(gcbh, 'IGainOutDataTypeStr')
      mask TypeOptions IProdOutDataTypeStr: I Gain/External Parameters/IProd Out/OutDataTypeStr
      mask Callback IProdOutDataTypeStr: pidpack.PIDConfig.callbackSyncDataType(gcbh, 'IProdOutDataTypeStr')
      mask TypeOptions IOutMin: I Gain/Internal Parameters/Integral Gain/OutMin | I Gain/External Parameters/IProd Out/OutMin
      mask TypeOptions IOutMax: I Gain/Internal Parameters/Integral Gain/OutMax | I Gain/External Parameters/IProd Out/OutMax
      mask TypeOptions DGainOutDataTypeStr: D Gain/Internal Parameters/Derivative Gain/OutDataTypeStr
      mask Callback DGainOutDataTypeStr: pidpack.PIDConfig.callbackSyncDataType(gcbh, 'DGainOutDataTypeStr')
      mask TypeOptions DProdOutDataTypeStr: D Gain/External Parameters/DProd Out/OutDataTypeStr
      mask Callback DProdOutDataTypeStr: pidpack.PIDConfig.callbackSyncDataType(gcbh, 'DProdOutDataTypeStr')
      mask TypeOptions DOutMin: D Gain/Internal Parameters/Derivative Gain/OutMin | D Gain/External Parameters/DProd Out/OutMin
      mask TypeOptions DOutMax: D Gain/Internal Parameters/Derivative Gain/OutMax | D Gain/External Parameters/DProd Out/OutMax
      mask TypeOptions NGainOutDataTypeStr: N Gain/Internal Parameters/Filter Coefficient/OutDataTypeStr
      mask Callback NGainOutDataTypeStr: pidpack.PIDConfig.callbackSyncDataType(gcbh, 'NGainOutDataTypeStr')
      mask TypeOptions NProdOutDataTypeStr: N Gain/External Parameters/NProd Out/OutDataTypeStr
      mask Callback NProdOutDataTypeStr: pidpack.PIDConfig.callbackSyncDataType(gcbh, 'NProdOutDataTypeStr')
      mask TypeOptions NOutMin: N Gain/Internal Parameters/Filter Coefficient/OutMin | N Gain/External Parameters/NProd Out/OutMin
      mask TypeOptions NOutMax: N Gain/Internal Parameters/Filter Coefficient/OutMax | N Gain/External Parameters/NProd Out/OutMax
      mask TypeOptions SumOutDataTypeStr: Sum Fdbk/Enabled/Sum Fdbk/OutDataTypeStr | Sum/Sum_PD/Sum/OutDataTypeStr | Sum/Sum_PI/Sum/OutDataTypeStr | Sum/Sum_PID/Sum/OutDataTypeStr
      mask TypeOptions SumOutMin: Sum Fdbk/Enabled/Sum Fdbk/OutMin | Sum/Sum_PD/Sum/OutMin | Sum/Sum_PI/Sum/OutMin | Sum/Sum_PID/Sum/OutMin
      mask TypeOptions SumOutMax: Sum Fdbk/Enabled/Sum Fdbk/OutMax | Sum/Sum_PD/Sum/OutMax | Sum/Sum_PI/Sum/OutMax | Sum/Sum_PID/Sum/OutMax
      mask TypeOptions SaturationOutDataTypeStr: Saturation/Enabled/Saturation/OutDataTypeStr | Saturation Fdbk/Enabled/Saturation/OutDataTypeStr
      mask TypeOptions SaturationOutMin:
      | Saturation/Enabled/Saturation/OutMin | Saturation Fdbk/Enabled/Saturation/OutMin | Saturation Fdbk/External/Saturation
      | Dynamic/OutMin | Saturation/External/Saturation
      | Dynamic/OutMin
      mask TypeOptions SaturationOutMax:
      | Saturation/Enabled/Saturation/OutMax | Saturation Fdbk/Enabled/Saturation/OutMax | Saturation/External/Saturation
      | Dynamic/OutMax | Saturation Fdbk/External/Saturation
      | Dynamic/OutMax
      mask TypeOptions PParamDataTypeStr: Ideal P Gain/Internal Parameters/Proportional Gain/ParamDataTypeStr | Ideal P Gain Fdbk/Internal Parameters/Proportional Gain/ParamDataTypeStr | Parallel P Gain/Internal Parameters/Proportional Gain/ParamDataTypeStr
      mask TypeOptions PParamMin: Ideal P Gain/Internal Parameters/Proportional Gain/ParamMin | Ideal P Gain Fdbk/Internal Parameters/Proportional Gain/ParamMin | Parallel P Gain/Internal Parameters/Proportional Gain/ParamMin
      mask TypeOptions PParamMax: Ideal P Gain/Internal Parameters/Proportional Gain/ParamMax | Ideal P Gain Fdbk/Internal Parameters/Proportional Gain/ParamMax | Parallel P Gain/Internal Parameters/Proportional Gain/ParamMax
      mask TypeOptions IParamDataTypeStr: I Gain/Internal Parameters/Integral Gain/ParamDataTypeStr
      mask TypeOptions IParamMin: I Gain/Internal Parameters/Integral Gain/ParamMin
      mask TypeOptions IParamMax: I Gain/Internal Parameters/Integral Gain/ParamMax
      mask TypeOptions DParamDataTypeStr: D Gain/Internal Parameters/Derivative Gain/ParamDataTypeStr
      mask TypeOptions DParamMin: D Gain/Internal Parameters/Derivative Gain/ParamMin
      mask TypeOptions DParamMax: D Gain/Internal Parameters/Derivative Gain/ParamMax
      mask TypeOptions NParamDataTypeStr: N Gain/Internal Parameters/Filter Coefficient/ParamDataTypeStr
      mask TypeOptions NParamMin: N Gain/Internal Parameters/Filter Coefficient/ParamMin
      mask TypeOptions NParamMax: N Gain/Internal Parameters/Filter Coefficient/ParamMax
      mask TypeOptions KbParamDataTypeStr: Anti-windup/Back Calculation/Kb/ParamDataTypeStr
      mask TypeOptions KbParamMin: Anti-windup/Back Calculation/Kb/ParamMin
      mask TypeOptions KbParamMax: Anti-windup/Back Calculation/Kb/ParamMax
      mask TypeOptions KtParamDataTypeStr: Tracking Mode/Enabled/Kt/ParamDataTypeStr
      mask TypeOptions KtParamMin: Tracking Mode/Enabled/Kt/ParamMin
      mask TypeOptions KtParamMax: Tracking Mode/Enabled/Kt/ParamMax
      mask TypeOptions KbOutDataTypeStr: Anti-windup/Back Calculation/Kb/OutDataTypeStr
      mask TypeOptions KbOutMin: Anti-windup/Back Calculation/Kb/OutMin
      mask TypeOptions KbOutMax: Anti-windup/Back Calculation/Kb/OutMax
      mask TypeOptions KtOutDataTypeStr: Tracking Mode/Enabled/Kt/OutDataTypeStr
      mask TypeOptions KtOutMin: Tracking Mode/Enabled/Kt/OutMin
      mask TypeOptions KtOutMax: Tracking Mode/Enabled/Kt/OutMax
      mask TypeOptions IntegratorOutDataTypeStr: Integrator/Discrete/Integrator/OutDataTypeStr
      mask TypeOptions IntegratorOutMin: Integrator/Discrete/Integrator/OutMin
      mask TypeOptions IntegratorOutMax: Integrator/Discrete/Integrator/OutMax
      mask TypeOptions FilterOutDataTypeStr: Filter/Disc. Forward Euler Filter/Filter/OutDataTypeStr
      mask TypeOptions FilterOutMin: Filter/Disc. Forward Euler Filter/Filter/OutMin
      mask TypeOptions FilterOutMax: Filter/Disc. Forward Euler Filter/Filter/OutMax
      mask TypeOptions SumI1OutDataTypeStr: Tracking Mode Sum/Tracking Mode/SumI1/OutDataTypeStr
      mask TypeOptions SumI1OutMin: Tracking Mode Sum/Tracking Mode/SumI1/OutMin
      mask TypeOptions SumI1OutMax: Tracking Mode Sum/Tracking Mode/SumI1/OutMax
      mask TypeOptions SumI2OutDataTypeStr: Anti-windup/Back Calculation/SumI2/OutDataTypeStr
      mask TypeOptions SumI2OutMin: Anti-windup/Back Calculation/SumI2/OutMin
      mask TypeOptions SumI2OutMax: Anti-windup/Back Calculation/SumI2/OutMax
      mask TypeOptions SumI3OutDataTypeStr: Tracking Mode/Enabled/SumI3/OutDataTypeStr
      mask TypeOptions SumI3OutMin: Tracking Mode/Enabled/SumI3/OutMin
      mask TypeOptions SumI3OutMax: Tracking Mode/Enabled/SumI3/OutMax
      mask TypeOptions SumI4OutDataTypeStr: Anti-windup/Back Calculation/SumI4/OutDataTypeStr
      mask TypeOptions SumI4OutMin: Anti-windup/Back Calculation/SumI4/OutMin
      mask TypeOptions SumI4OutMax: Anti-windup/Back Calculation/SumI4/OutMax
      mask TypeOptions SumDOutDataTypeStr: Filter/Cont. Filter/SumD/OutDataTypeStr | Filter/Disc. Forward Euler Filter/SumD/OutDataTypeStr
      mask TypeOptions SumDOutMin: Filter/Cont. Filter/SumD/OutMin | Filter/Disc. Forward Euler Filter/SumD/OutMin
      mask TypeOptions SumDOutMax: Filter/Cont. Filter/SumD/OutMax | Filter/Disc. Forward Euler Filter/SumD/OutMax
      mask TypeOptions SumAccumDataTypeStr: Sum Fdbk/Enabled/Sum Fdbk/AccumDataTypeStr | Sum/Sum_PD/Sum/AccumDataTypeStr | Sum/Sum_PI/Sum/AccumDataTypeStr | Sum/Sum_PID/Sum/AccumDataTypeStr
      mask TypeOptions SumI1AccumDataTypeStr: Tracking Mode Sum/Tracking Mode/SumI1/AccumDataTypeStr
      mask TypeOptions SumI2AccumDataTypeStr: Anti-windup/Back Calculation/SumI2/AccumDataTypeStr
      mask TypeOptions SumI3AccumDataTypeStr: Tracking Mode/Enabled/SumI3/AccumDataTypeStr
      mask TypeOptions SumI4AccumDataTypeStr: Anti-windup/Back Calculation/SumI4/AccumDataTypeStr
      mask TypeOptions SumDAccumDataTypeStr: Filter/Cont. Filter/SumD/AccumDataTypeStr | Filter/Disc. Forward Euler Filter/SumD/AccumDataTypeStr
      mask TypeOptions FilterDiffNumProductOutputDataTypeStr: Filter/Disc. Backward Euler Filter/Filter Differentiator TF/NumProductDataTypeStr | Filter/Disc. Trapezoidal Filter/Filter Differentiator TF/NumProductDataTypeStr
      mask TypeOptions FilterDiffDenProductOutputDataTypeStr: Filter/Disc. Backward Euler Filter/Filter Differentiator TF/DenProductDataTypeStr | Filter/Disc. Trapezoidal Filter/Filter Differentiator TF/DenProductDataTypeStr
      mask TypeOptions FilterDiffNumAccumDataTypeStr: Filter/Disc. Backward Euler Filter/Filter Differentiator TF/NumAccumDataTypeStr | Filter/Disc. Trapezoidal Filter/Filter Differentiator TF/NumAccumDataTypeStr
      mask TypeOptions FilterDiffDenAccumDataTypeStr: Filter/Disc. Backward Euler Filter/Filter Differentiator TF/DenAccumDataTypeStr | Filter/Disc. Trapezoidal Filter/Filter Differentiator TF/DenAccumDataTypeStr
      mask TypeOptions FilterDiffOutCoefDataTypeStr: Filter/Disc. Backward Euler Filter/DenCoefOut/OutDataTypeStr | Filter/Disc. Trapezoidal Filter/DenCoefOut/OutDataTypeStr
      mask TypeOptions FilterDiffOutCoefMin: Filter/Disc. Backward Euler Filter/DenCoefOut/OutMin | Filter/Disc. Trapezoidal Filter/DenCoefOut/OutMin
      mask TypeOptions FilterDiffOutCoefMax: Filter/Disc. Backward Euler Filter/DenCoefOut/OutMax | Filter/Disc. Trapezoidal Filter/DenCoefOut/OutMax
      mask TypeOptions ReciprocalOutDataTypeStr: Filter/Disc. Backward Euler Filter/Reciprocal/OutDataTypeStr | Filter/Disc. Trapezoidal Filter/Reciprocal/OutDataTypeStr
      mask TypeOptions ReciprocalOutMin: Filter/Disc. Backward Euler Filter/Reciprocal/OutMin | Filter/Disc. Trapezoidal Filter/Reciprocal/OutMin
      mask TypeOptions ReciprocalOutMax: Filter/Disc. Backward Euler Filter/Reciprocal/OutMax | Filter/Disc. Trapezoidal Filter/Reciprocal/OutMax
      mask TypeOptions SumDenOutDataTypeStr: Filter/Disc. Backward Euler Filter/SumDen/OutDataTypeStr | Filter/Disc. Trapezoidal Filter/SumDen/OutDataTypeStr
      mask TypeOptions SumDenOutMin: Filter/Disc. Backward Euler Filter/SumDen/OutMin | Filter/Disc. Trapezoidal Filter/SumDen/OutMin
      mask TypeOptions SumDenOutMax: Filter/Disc. Backward Euler Filter/SumDen/OutMax | Filter/Disc. Trapezoidal Filter/SumDen/OutMax
      mask TypeOptions SumNumOutDataTypeStr: Filter/Disc. Trapezoidal Filter/SumNum/OutDataTypeStr
      mask TypeOptions SumNumOutMin: Filter/Disc. Trapezoidal Filter/SumNum/OutMin
      mask TypeOptions SumNumOutMax: Filter/Disc. Trapezoidal Filter/SumNum/OutMax
      mask TypeOptions SumDenAccumDataTypeStr: Filter/Disc. Backward Euler Filter/SumDen/AccumDataTypeStr | Filter/Disc. Trapezoidal Filter/SumDen/AccumDataTypeStr
      mask TypeOptions SumNumAccumDataTypeStr: Filter/Disc. Trapezoidal Filter/SumNum/AccumDataTypeStr
      mask TypeOptions DivideOutDataTypeStr: Filter/Disc. Trapezoidal Filter/Divide/OutDataTypeStr
      mask TypeOptions DivideOutMin: Filter/Disc. Trapezoidal Filter/Divide/OutMin
      mask TypeOptions DivideOutMax: Filter/Disc. Trapezoidal Filter/Divide/OutMax
      mask TypeOptions UdiffTsProdOutDataTypeStr: Filter/Differentiator/Tsamp/External Ts/Udiff*Ts Prod Out/OutDataTypeStr
      mask TypeOptions UdiffTsProdOutMin: Filter/Differentiator/Tsamp/External Ts/Udiff*Ts Prod Out/OutMin
      mask TypeOptions UdiffTsProdOutMax: Filter/Differentiator/Tsamp/External Ts/Udiff*Ts Prod Out/OutMax
      mask TypeOptions NTsProdOutDataTypeStr: Filter/Disc. Backward Euler Filter/Tsamp/External Ts/N*Ts Prod Out/OutDataTypeStr | Filter/Disc. Trapezoidal Filter/Tsamp/External Ts/N*Ts Prod Out/OutDataTypeStr
      mask TypeOptions NTsProdOutMin: Filter/Disc. Backward Euler Filter/Tsamp/External Ts/N*Ts Prod Out/OutMin | Filter/Disc. Trapezoidal Filter/Tsamp/External Ts/N*Ts Prod Out/OutMin
      mask TypeOptions NTsProdOutMax: Filter/Disc. Backward Euler Filter/Tsamp/External Ts/N*Ts Prod Out/OutMax | Filter/Disc. Trapezoidal Filter/Tsamp/External Ts/N*Ts Prod Out/OutMax
      mask TypeOptions UintegralTsProdOutDataTypeStr: Tsamp - Integral/External Ts/Uintegral*Ts Prod Out/OutDataTypeStr
      mask TypeOptions UintegralTsProdOutMin: Tsamp - Integral/External Ts/Uintegral*Ts Prod Out/OutMin
      mask TypeOptions UintegralTsProdOutMax: Tsamp - Integral/External Ts/Uintegral*Ts Prod Out/OutMax
      mask TypeOptions UngainTsProdOutDataTypeStr: Tsamp - Ngain/External Ts/Ungain*Ts Prod Out/OutDataTypeStr
      mask TypeOptions UngainTsProdOutMin: Tsamp - Ngain/External Ts/Ungain*Ts Prod Out/OutMin
      mask TypeOptions UngainTsProdOutMax: Tsamp - Ngain/External Ts/Ungain*Ts Prod Out/OutMax
      mask TypeOptions ClampingZeroOutDataTypeStr: Anti-windup/Disc. Clamping Ideal/Clamping_zero/OutDataTypeStr | Anti-windup/Disc. Clamping Parallel/Clamping_zero/OutDataTypeStr
      mask TypeOptions ClampingZeroOutMin: Anti-windup/Disc. Clamping Ideal/Clamping_zero/OutMin | Anti-windup/Disc. Clamping Parallel/Clamping_zero/OutMin
      mask TypeOptions ClampingZeroOutMax: Anti-windup/Disc. Clamping Ideal/Clamping_zero/OutMax | Anti-windup/Disc. Clamping Parallel/Clamping_zero/OutMax
      mask TypeOptions FilterDenConstantOutDataTypeStr: Filter/Disc. Backward Euler Filter/Filter Den Constant/OutDataTypeStr | Filter/Disc. Trapezoidal Filter/Filter Den Constant/OutDataTypeStr
      mask TypeOptions FilterDenConstantOutMin: Filter/Disc. Backward Euler Filter/Filter Den Constant/OutMin | Filter/Disc. Trapezoidal Filter/Filter Den Constant/OutMin
      mask TypeOptions FilterDenConstantOutMax: Filter/Disc. Backward Euler Filter/Filter Den Constant/OutMax | Filter/Disc. Trapezoidal Filter/Filter Den Constant/OutMax
      mask TypeOptions PCopyOutDataTypeStr: P Copy/Internal Parameters Ideal/P Copy/OutDataTypeStr
      mask TypeOptions PCopyOutMin: P Copy/Internal Parameters Ideal/P Copy/OutMin
      mask TypeOptions PCopyOutMax: P Copy/Internal Parameters Ideal/P Copy/OutMax
      mask TypeOptions NCopyOutDataTypeStr: N Copy/Internal Parameters/N Copy/OutDataTypeStr
      mask TypeOptions NCopyOutMin: N Copy/Internal Parameters/N Copy/OutMin
      mask TypeOptions NCopyOutMax: N Copy/Internal Parameters/N Copy/OutMax
      mask TypeOptions IntegratorContinuousStateAttributes: Integrator/Continuous/Integrator/ContinuousStateAttributes
      mask TypeOptions IntegratorStateIdentifier: Integrator/Discrete/Integrator/StateName
      mask Callback IntegratorStateIdentifier: pidpack.PIDConfig.callbackStateAttributes(gcbh,'Integrator')
      mask Callback IntegratorStateMustResolveToSignalObject: pidpack.PIDConfig.callbackStateAttributes(gcbh,'Integrator')
      mask TypeOptions IntegratorRTWStateStorageClass: Simulink:masks:Auto | Simulink:masks:ExportedGlobal | Simulink:masks:ImportedExtern | Simulink:masks:ImportedExternPointer
      mask TypeOptions FilterContinuousStateAttributes: Filter/Cont. Filter/Filter/ContinuousStateAttributes
      mask TypeOptions FilterStateIdentifier: Filter/Disc. Backward Euler Filter/Filter Differentiator TF/StateName | Filter/Disc. Forward Euler Filter/Filter/StateName | Filter/Disc. Trapezoidal Filter/Filter Differentiator TF/StateName
      mask Callback FilterStateIdentifier: pidpack.PIDConfig.callbackStateAttributes(gcbh,'Filter')
      mask Callback FilterStateMustResolveToSignalObject: pidpack.PIDConfig.callbackStateAttributes(gcbh,'Filter')
      mask TypeOptions FilterRTWStateStorageClass: Simulink:masks:Auto | Simulink:masks:ExportedGlobal | Simulink:masks:ImportedExtern | Simulink:masks:ImportedExternPointer
      mask TypeOptions ParallelPVariant: Parallel P Gain/LabelModeActiveChoice
      mask TypeOptions IdealPVariant: Ideal P Gain/LabelModeActiveChoice
      mask TypeOptions IVariant: I Gain/LabelModeActiveChoice
      mask TypeOptions DVariant: D Gain/LabelModeActiveChoice
      mask TypeOptions IntegratorVariant: Integrator/LabelModeActiveChoice
      mask TypeOptions SatVariant: Saturation/LabelModeActiveChoice | Anti-windup/Disc. Clamping Parallel/Dead Zone/LabelModeActiveChoice | Anti-windup/Cont. Clamping Ideal/Dead Zone/LabelModeActiveChoice | Anti-windup/Cont. Clamping Parallel/Dead Zone/LabelModeActiveChoice | Anti-windup/Disc. Clamping Ideal/Dead Zone/LabelModeActiveChoice
      mask TypeOptions AWVariant: Anti-windup/LabelModeActiveChoice
      mask TypeOptions PCopyVariant: P Copy/LabelModeActiveChoice
      mask TypeOptions TRVariant: Tracking Mode/LabelModeActiveChoice
      mask TypeOptions FdbkBlocksVariant: postSat Signal/LabelModeActiveChoice | preSat Signal/LabelModeActiveChoice
      mask TypeOptions IdealPFdbkVariant: Ideal P Gain Fdbk/LabelModeActiveChoice
      mask TypeOptions SatFdbkVariant: Saturation Fdbk/LabelModeActiveChoice
      mask TypeOptions DerivativeFilterVariant: Filter/LabelModeActiveChoice
      mask TypeOptions NVariant: N Gain/LabelModeActiveChoice
      mask TypeOptions NCopyVariant: N Copy/LabelModeActiveChoice
      mask TypeOptions FilterICVariant: Filter ICs/LabelModeActiveChoice
      mask TypeOptions IntegratorICVariant: Integrator ICs/LabelModeActiveChoice
      mask TypeOptions ExternalResetVariant: Reset Signal/LabelModeActiveChoice
      mask TypeOptions TRSumVariant: Tracking Mode Sum/LabelModeActiveChoice
      mask TypeOptions SumFdbkVariant: Sum Fdbk/LabelModeActiveChoice
      mask TypeOptions SumVariant: Sum/LabelModeActiveChoice
      mask TypeOptions TsampFilterVariant: Filter/Disc. Backward Euler Filter/Tsamp/LabelModeActiveChoice | Filter/Disc. Trapezoidal Filter/Tsamp/LabelModeActiveChoice | Filter/Differentiator/Tsamp/LabelModeActiveChoice
      mask TypeOptions TsampNgainVariant: Tsamp - Ngain/LabelModeActiveChoice
      mask TypeOptions TsampIntegralVariant: Tsamp - Integral/LabelModeActiveChoice
      mask TypeOptions ExternalSaturationOutDataTypeStr:
      | Saturation/External/Saturation
      | Dynamic/OutDataTypeStr | Saturation Fdbk/External/Saturation
      | Dynamic/OutDataTypeStr
      mask TypeOptions DerivativeSourceVariant: External Derivative/LabelModeActiveChoice
      mask TypeOptions InitialConditionSetting: Integrator/Discrete/Integrator/InitialConditionSetting | Filter/Disc. Forward Euler Filter/Filter/InitialConditionSetting | Anti-windup/Cont. Clamping Ideal/Memory/InitialConditionSetting | Anti-windup/Cont. Clamping Parallel/Memory/InitialConditionSetting | Filter/Cont. Filter/Filter/InitialConditionSetting | Filter/Differentiator/UD/InitialConditionSetting | Integrator/Continuous/Integrator/InitialConditionSetting
      mask TypeOptions PreIntVariant: preInt Signal/LabelModeActiveChoice
      mask DialogControl Controller Prompt: Controller:
      mask DialogControl Form Prompt: Form:
      mask DialogControl TimeDomain Prompt: Time domain:
      mask DialogControl grpDiscrete Prompt: Simulink:masks:DiscreteTimeSettings_GT
      mask DialogControl UseExternalTs Prompt: PID Controller is inside a conditionally executed subsystem
      mask DialogControl SampleTime Prompt: Sample time (-1 for inherited):
      mask DialogControl grpIntFiltMethod Prompt: Simulink:masks:IntFiltMethods_GT
      mask DialogControl IntegratorMethod Prompt: Integrator method:
      mask DialogControl FilterMethod Prompt: Filter method:
      mask DialogControl grpCompensatorFormula Prompt: Simulink:masks:PIDCompensatorFormula
      mask DialogControl tabMain Prompt: Simulink:masks:Main
      mask DialogControl grpControlParameters Prompt: Simulink:masks:ControllerParameters_GT
      mask DialogControl ControllerParametersSource Prompt: Source:
      mask DialogControl P Prompt: Proportional (P):
      mask DialogControl I Prompt: Integral (I):
      mask DialogControl UseKiTs Prompt: Use I*Ts (optimal for codegen)
      mask DialogControl D Prompt: Derivative (D):
      mask DialogControl UseExternalDerivativeSource Prompt: Use externally sourced derivative
      mask DialogControl N Prompt: Filter coefficient (N):
      mask DialogControl UseFilter Prompt: Use filtered derivative
      mask DialogControl grpAutoTune Prompt: Simulink:masks:AutomatedTuning_GT
      mask DialogControl TunerSelectOption Prompt: Select tuning method:
      mask DialogControl TuneButton Prompt: Simulink:masks:PIDTune
      mask DialogControl TuneButton Callback: pidpack.PIDConfig.callbackTuneButton(gcbh)
      mask DialogControl ZeroCross Prompt: Enable zero-crossing detection
      mask DialogControl tabInitialization Prompt: Simulink:masks:Initialization_TAB
      mask DialogControl txtNoInitializationTab Prompt: Simulink:masks:InitializationEmptyTab_GT
      mask DialogControl grpInitialConditions Prompt: Simulink:masks:IntegratorFilterInitialConditions_GT
      mask DialogControl InitialConditionSource Prompt: Source:
      mask DialogControl InitialConditionForIntegrator Prompt: Integrator:
      mask DialogControl InitialConditionForFilter Prompt: Filter:
      mask DialogControl DifferentiatorICPrevScaledInput Prompt: Differentiator:
      mask DialogControl grpExternalReset Prompt: Simulink:masks:ExternalReset_MP
      mask DialogControl ExternalReset Prompt: External reset:
      mask DialogControl IgnoreLimit Prompt: Ignore reset when linearizing
      mask DialogControl grpTracking Prompt: Simulink:masks:TrackingMode_GT
      mask DialogControl TrackingMode Prompt: Enable tracking mode
      mask DialogControl Kt Prompt: Tracking coefficient (Kt):
      mask DialogControl tabOutputSaturation Prompt: Simulink:masks:OutputSaturation_TAB
      mask DialogControl grpOutputSaturation Prompt: Simulink:masks:OutputSaturation_GT
      mask DialogControl LimitOutput Prompt: Limit output
      mask DialogControl SatLimitsSource Prompt: Source:
      mask DialogControl UpperSaturationLimit Prompt: Upper limit:
      mask DialogControl LowerSaturationLimit Prompt: Lower limit:
      mask DialogControl LinearizeAsGain Prompt: Ignore saturation when linearizing
      mask DialogControl grpAntiWindup Prompt: Simulink:masks:AntiwindupMethod_GT
      mask DialogControl AntiWindupMode Prompt: Anti-windup Method:
      mask DialogControl Kb Prompt: Back-calculation coefficient (Kb):
      mask DialogControl grpIntegratorSaturation Prompt: Simulink:masks:IntegratorSaturation_GT
      mask DialogControl LimitIntegrator Prompt: Limit output
      mask DialogControl UpperIntegratorSaturationLimit Prompt: Upper limit:
      mask DialogControl LowerIntegratorSaturationLimit Prompt: Lower limit:
      mask DialogControl tabDataTypes Prompt: Simulink:dialog:DataTypesTab
      mask DialogControl tabFixedPointOpParams Prompt: Simulink:masks:FixedPointOperationalParameters_GT
      mask DialogControl RndMeth Prompt: Integer rounding mode:
      mask DialogControl SaturateOnIntegerOverflow Prompt: Saturate on integer overflow
      mask DialogControl LockScale Prompt: Lock data type settings against changes by the fixed-point tools
      mask DialogControl btnFixedPointTool Prompt: Simulink:masks:FixedPointToolBtn
      mask DialogControl btnFixedPointTool Callback: pidpack.PIDConfig.callbackFixedPointButton(gcbh)
      mask DialogControl txtDataType Prompt: Simulink:dialog:DataTypeColumnLabel
      mask DialogControl txtMinimum Prompt: Simulink:dialog:MinimumColumnLabel
      mask DialogControl txtMaximum Prompt: Simulink:dialog:MaximumColumnLabel
      mask DialogControl PGainOutDataTypeStr Prompt: P product output:
      mask DialogControl PProdOutDataTypeStr Prompt: P product output:
      mask DialogControl IGainOutDataTypeStr Prompt: I product output:
      mask DialogControl IProdOutDataTypeStr Prompt: I product output:
      mask DialogControl DGainOutDataTypeStr Prompt: D product output:
      mask DialogControl DProdOutDataTypeStr Prompt: D product output:
      mask DialogControl NGainOutDataTypeStr Prompt: N product output:
      mask DialogControl NProdOutDataTypeStr Prompt: N product output:
      mask DialogControl SumOutDataTypeStr Prompt: Sum output:
      mask DialogControl SaturationOutDataTypeStr Prompt: Saturation output:
      mask DialogControl grpExtraDataTypes Prompt: Simulink:masks:AdditionalDataTypes_GT
      mask DialogControl txtDataType_2 Prompt: Simulink:dialog:DataTypeColumnLabel
      mask DialogControl txtMinimum_2 Prompt: Simulink:dialog:MinimumColumnLabel
      mask DialogControl txtMaximum_2 Prompt: Simulink:dialog:MaximumColumnLabel
      mask DialogControl PParamDataTypeStr Prompt: P parameter:
      mask DialogControl IParamDataTypeStr Prompt: I parameter:
      mask DialogControl DParamDataTypeStr Prompt: D parameter:
      mask DialogControl NParamDataTypeStr Prompt: N parameter:
      mask DialogControl KbParamDataTypeStr Prompt: Kb parameter:
      mask DialogControl KtParamDataTypeStr Prompt: Kt parameter:
      mask DialogControl KbOutDataTypeStr Prompt: Kb product output:
      mask DialogControl KtOutDataTypeStr Prompt: Kt product output:
      mask DialogControl IntegratorOutDataTypeStr Prompt: Integrator output:
      mask DialogControl FilterOutDataTypeStr Prompt: Filter output:
      mask DialogControl SumI1OutDataTypeStr Prompt: SumI1 output:
      mask DialogControl SumI2OutDataTypeStr Prompt: SumI2 output:
      mask DialogControl SumI3OutDataTypeStr Prompt: SumI3 output:
      mask DialogControl SumI4OutDataTypeStr Prompt: SumI4 output:
      mask DialogControl SumDOutDataTypeStr Prompt: SumD output:
      mask DialogControl SumAccumDataTypeStr Prompt: Accumulator of Sum:
      mask DialogControl SumI1AccumDataTypeStr Prompt: Accumulator of SumI1:
      mask DialogControl SumI2AccumDataTypeStr Prompt: Accumulator of SumI2:
      mask DialogControl SumI3AccumDataTypeStr Prompt: Accumulator of SumI3:
      mask DialogControl SumI4AccumDataTypeStr Prompt: Accumulator of SumI4:
      mask DialogControl SumDAccumDataTypeStr Prompt: Accumulator of SumD:
      mask DialogControl DifferentiatorOutDataTypeStr Prompt: Differentiator output:
      mask DialogControl FilterDiffNumProductOutputDataTypeStr Prompt: Filter Numerator product output:
      mask DialogControl FilterDiffDenProductOutputDataTypeStr Prompt: Filter Denominator product output:
      mask DialogControl FilterDiffNumAccumDataTypeStr Prompt: Filter Numerator accumulator:
      mask DialogControl FilterDiffDenAccumDataTypeStr Prompt: Filter Denominator accumulator:
      mask DialogControl FilterDiffOutCoefDataTypeStr Prompt: Filter Coefficient product output:
      mask DialogControl ReciprocalOutDataTypeStr Prompt: Reciprocal output:
      mask DialogControl SumDenOutDataTypeStr Prompt: SumDen output:
      mask DialogControl SumNumOutDataTypeStr Prompt: SumNum output:
      mask DialogControl SumDenAccumDataTypeStr Prompt: Accumulator of SumDen:
      mask DialogControl SumNumAccumDataTypeStr Prompt: Accumulator of SumNum:
      mask DialogControl DivideOutDataTypeStr Prompt: Divide output:
      mask DialogControl UdiffTsProdOutDataTypeStr Prompt: U_differentiator * Ts Product Out:
      mask DialogControl NTsProdOutDataTypeStr Prompt: N * Ts product output:
      mask DialogControl UintegralTsProdOutDataTypeStr Prompt: U_integral * Ts product output:
      mask DialogControl UngainTsProdOutDataTypeStr Prompt: U_Ngain * Ts product output:
      mask DialogControl ClampingZeroOutDataTypeStr Prompt: Clamping algorithm constant zero (Clamping_zero) output:
      mask DialogControl FilterDenConstantOutDataTypeStr Prompt: Filter coefficient denominator constant (Filter Den Constant) output:
      mask DialogControl PCopyOutDataTypeStr Prompt: P Parameter constant (Pcopy) output:
      mask DialogControl NCopyOutDataTypeStr Prompt: N Parameter constant (Ncopy) output:
      mask DialogControl tabStateAttributes Prompt: Simulink:dialog:StateAttributes
      mask DialogControl txtNoStateTab Prompt: Simulink:masks:StateAttributesEmptyTab_GT
      mask DialogControl grpIntegratorState Prompt: Simulink:masks:IntegratorState_GT
      mask DialogControl IntegratorContinuousStateAttributes Prompt: State name: (e.g., 'position')
      mask DialogControl IntegratorStateIdentifier Prompt: State name:
      mask DialogControl IntegratorStateMustResolveToSignalObject Prompt: State name must resolve to Simulink signal object
      mask DialogControl IntegratorRTWStateStorageClass Prompt: Code generation storage class:
      mask DialogControl IntegratorRTWStateStorageTypeQualifier Prompt: Code generation storage type qualifier:
      mask DialogControl grpFilterState Prompt: Simulink:masks:FilterState_GT
      mask DialogControl FilterContinuousStateAttributes Prompt: State name: (e.g., 'position')
      mask DialogControl FilterStateIdentifier Prompt: State name:
      mask DialogControl FilterStateMustResolveToSignalObject Prompt: State name must resolve to Simulink signal object
      mask DialogControl FilterRTWStateStorageClass Prompt: Code generation storage class:
      mask DialogControl FilterRTWStateStorageTypeQualifier Prompt: Code generation storage type qualifier:
      mask DialogControl grpVariants Prompt: Hidden Parameters
      mask DialogControl ParallelPVariant Prompt: Variant:
      mask DialogControl IdealPVariant Prompt: Variant:
      mask DialogControl IVariant Prompt: Variant:
      mask DialogControl DVariant Prompt: Variant:
      mask DialogControl IntegratorVariant Prompt: Variant:
      mask DialogControl SatVariant Prompt: Variant:
      mask DialogControl AWVariant Prompt: Variant:
      mask DialogControl PCopyVariant Prompt: Variant:
      mask DialogControl TRVariant Prompt: Variant:
      mask DialogControl FdbkBlocksVariant Prompt: Variant:
      mask DialogControl IdealPFdbkVariant Prompt: Variant:
      mask DialogControl SatFdbkVariant Prompt: Variant:
      mask DialogControl DerivativeFilterVariant Prompt: Variant:
      mask DialogControl NVariant Prompt: Variant:
      mask DialogControl NCopyVariant Prompt: Variant:
      mask DialogControl FilterICVariant Prompt: Variant:
      mask DialogControl IntegratorICVariant Prompt: Variant:
      mask DialogControl ExternalResetVariant Prompt: Variant:
      mask DialogControl TRSumVariant Prompt: Variant:
      mask DialogControl SumFdbkVariant Prompt: Variant:
      mask DialogControl SumVariant Prompt: Variant:
      mask DialogControl TsampFilterVariant Prompt: Label mode active choice:
      mask DialogControl TsampNgainVariant Prompt: Label mode active choice:
      mask DialogControl TsampIntegralVariant Prompt: Label mode active choice:
      mask DialogControl ExternalSaturationOutDataTypeStr Prompt: Saturation output:
      mask DialogControl DerivativeSourceVariant Prompt: Label mode active choice:
      mask DialogControl InitialConditionSetting Prompt: Initial condition setting:
      mask DialogControl PreIntVariant Prompt: Label mode active choice:
      mask Display:
      | iconstr = pidpack.PIDConfig.utilGetMaskDisplayString(gcbh);
      | eval(iconstr)
  Discrete Transfer Fcn : DiscreteTransferFcn  Numerator=[0.00995017]  Denominator=[1 -0.99004983]
  Droop_LPF : DiscreteTransferFcn  Numerator=[1-a_lpf_sys]  Denominator=[1 -a_lpf_sys]  SampleTime=Tsw
  Droop_Rd : Gain  Gain=Rd_bat
  Droop_Sum : Sum  Inputs=|+-
  Error_Sum : Sum  Inputs=|+-
  Error_Sum1 : Sum  Inputs=|+-
  G_canCh : Relay  OnSwitchValue=socLimit.max  OffSwitchValue=socLimit.rechargeBelow  OnOutputValue=0  OffOutputValue=1
  G_canDis : Relay  OnSwitchValue=socLimit.dischargeAbove  OffSwitchValue=socLimit.min
  G_ch : DataTypeConversion  OutDataTypeStr=double  SaturateOnIntegerOverflow=off  RndMeth=Floor
  G_dis : DataTypeConversion  OutDataTypeStr=double  SaturateOnIntegerOverflow=off  RndMeth=Floor
  G_loI : Gain  Gain=-thetaMaxDab
  G_loV : Gain  Gain=-45
  G_upI : Gain  Gain=thetaMaxDab
  G_upV : Gain  Gain=45
  PIctrl : Subsystem  AncestorBlock=mcblib/Control/Synchronous Machine/Controllers/PI Controller  mask(PID 1dof){Controller=PI, Form=Parallel, TimeDomain=Discrete-time, UseExternalTs=off, SampleTime=Tsw, IntegratorMethod=Forward Euler, FilterMethod=Forward Euler, ControllerParametersSource=internal, P=kpVoltage, I=kiVoltage, UseKiTs=off, D=0, UseExternalDerivativeSource=off, N=100, UseFilter=on, TunerSelectOption=Transfer Function Based (PID Tuner App), ZeroCross=on, InitialConditionSource=internal, InitialConditionForIntegrator=thetaIC, InitialConditionForFilter=0, DifferentiatorICPrevScaledInput=0, ExternalReset=none, IgnoreLimit=off, TrackingMode=off, Kt=1, LimitOutput=on, SatLimitsSource=external, UpperSaturationLimit=45, LowerSaturationLimit=-45, LinearizeAsGain=off, AntiWindupMode=clamping, Kb=1, LimitIntegrator=off, UpperIntegratorSaturationLimit=inf, LowerIntegratorSaturationLimit=-inf, RndMeth=Simplest, SaturateOnIntegerOverflow=off, LockScale=off, PGainOutDataTypeStr=Inherit: Same as input, PProdOutDataTypeStr=Inherit: Same as first input, POutMin=[], POutMax=[], IGainOutDataTypeStr=Inherit: Same as input, IProdOutDataTypeStr=Inherit: Same as first input, IOutMin=[], IOutMax=[], DGainOutDataTypeStr=Inherit: Inherit via internal rule, DProdOutDataTypeStr=Inherit: Inherit via internal rule, DOutMin=[], DOutMax=[], NGainOutDataTypeStr=Inherit: Inherit via internal rule, NProdOutDataTypeStr=Inherit: Inherit via internal rule, NOutMin=[], NOutMax=[], SumOutDataTypeStr=Inherit: Same as first input, SumOutMin=[], SumOutMax=[], SaturationOutDataTypeStr=Inherit: Inherit via back propagation, SaturationOutMin=[], SaturationOutMax=[], PParamDataTypeStr=Inherit: Inherit via internal rule, PParamMin=[], PParamMax=[], IParamDataTypeStr=Inherit: Inherit via internal rule, IParamMin=[], IParamMax=[], DParamDataTypeStr=Inherit: Inherit via internal rule, DParamMin=[], DParamMax=[], NParamDataTypeStr=Inherit: Inherit via internal rule, NParamMin=[], NParamMax=[], KbParamDataTypeStr=Inherit: Inherit via internal rule, KbParamMin=[], KbParamMax=[], KtParamDataTypeStr=Inherit: Inherit via internal rule, KtParamMin=[], KtParamMax=[], KbOutDataTypeStr=Inherit: Inherit via internal rule, KbOutMin=[], KbOutMax=[], KtOutDataTypeStr=Inherit: Inherit via internal rule, KtOutMin=[], KtOutMax=[], IntegratorOutDataTypeStr=Inherit: Inherit via internal rule, IntegratorOutMin=[], IntegratorOutMax=[], FilterOutDataTypeStr=Inherit: Inherit via internal rule, FilterOutMin=[], FilterOutMax=[], SumI1OutDataTypeStr=Inherit: Inherit via internal rule, SumI1OutMin=[], SumI1OutMax=[], SumI2OutDataTypeStr=Inherit: Inherit via internal rule, SumI2OutMin=[], SumI2OutMax=[], SumI3OutDataTypeStr=Inherit: Inherit via internal rule, SumI3OutMin=[], SumI3OutMax=[], SumI4OutDataTypeStr=Inherit: Inherit via internal rule, SumI4OutMin=[], SumI4OutMax=[], SumDOutDataTypeStr=Inherit: Inherit via internal rule, SumDOutMin=[], SumDOutMax=[], SumAccumDataTypeStr=Inherit: Inherit via internal rule, SumI1AccumDataTypeStr=Inherit: Inherit via internal rule, SumI2AccumDataTypeStr=Inherit: Inherit via internal rule, SumI3AccumDataTypeStr=Inherit: Inherit via internal rule, SumI4AccumDataTypeStr=Inherit: Inherit via internal rule, SumDAccumDataTypeStr=Inherit: Inherit via internal rule, DifferentiatorOutDataTypeStr=Inherit: Inherit via internal rule, DifferentiatorOutMin=[], DifferentiatorOutMax=[], FilterDiffNumProductOutputDataTypeStr=Inherit: Inherit via internal rule, FilterDiffDenProductOutputDataTypeStr=Inherit: Inherit via internal rule, FilterDiffNumAccumDataTypeStr=Inherit: Inherit via internal rule, FilterDiffDenAccumDataTypeStr=Inherit: Inherit via internal rule, FilterDiffOutCoefDataTypeStr=Inherit: Inherit via internal rule, FilterDiffOutCoefMin=[], FilterDiffOutCoefMax=[], ReciprocalOutDataTypeStr=Inherit: Inherit via internal rule, ReciprocalOutMin=[], ReciprocalOutMax=[], SumDenOutDataTypeStr=Inherit: Inherit via internal rule, SumDenOutMin=[], SumDenOutMax=[], SumNumOutDataTypeStr=Inherit: Inherit via internal rule, SumNumOutMin=[], SumNumOutMax=[], SumDenAccumDataTypeStr=Inherit: Inherit via internal rule, SumNumAccumDataTypeStr=Inherit: Inherit via internal rule, DivideOutDataTypeStr=Inherit: Inherit via internal rule, DivideOutMin=[], DivideOutMax=[], UdiffTsProdOutDataTypeStr=Inherit: Inherit via internal rule, UdiffTsProdOutMin=[], UdiffTsProdOutMax=[], NTsProdOutDataTypeStr=Inherit: Inherit via internal rule, NTsProdOutMin=[], NTsProdOutMax=[], UintegralTsProdOutDataTypeStr=Inherit: Inherit via internal rule, UintegralTsProdOutMin=[], UintegralTsProdOutMax=[], UngainTsProdOutDataTypeStr=Inherit: Inherit via internal rule, UngainTsProdOutMin=[], UngainTsProdOutMax=[], ClampingZeroOutDataTypeStr=Inherit: Inherit via back propagation, ClampingZeroOutMin=[], ClampingZeroOutMax=[], FilterDenConstantOutDataTypeStr=Inherit: Inherit via back propagation, FilterDenConstantOutMin=[], FilterDenConstantOutMax=[], PCopyOutDataTypeStr=Inherit: Inherit via back propagation, PCopyOutMin=[], PCopyOutMax=[], NCopyOutDataTypeStr=Inherit: Inherit via back propagation, NCopyOutMin=[], NCopyOutMax=[], IntegratorContinuousStateAttributes='', IntegratorStateIdentifier=, IntegratorStateMustResolveToSignalObject=off, IntegratorRTWStateStorageClass=Auto, IntegratorRTWStateStorageTypeQualifier=, FilterContinuousStateAttributes='', FilterStateIdentifier=, FilterStateMustResolveToSignalObject=off, FilterRTWStateStorageClass=Auto, FilterRTWStateStorageTypeQualifier=, ParallelPVariant=InternalParameters, IdealPVariant=Disabled, IVariant=InternalParameters, DVariant=Disabled, IntegratorVariant=Discrete, SatVariant=External, AWVariant=DiscClampingParallel, PCopyVariant=Disabled, TRVariant=Disabled, FdbkBlocksVariant=Forward, IdealPFdbkVariant=Disabled, SatFdbkVariant=Disabled, DerivativeFilterVariant=Disabled, NVariant=Disabled, NCopyVariant=Disabled_SignalSpec, FilterICVariant=Disabled, IntegratorICVariant=InternalICs, ExternalResetVariant=Disabled, TRSumVariant=Passthrough, SumFdbkVariant=Disabled, SumVariant=Sum_PI, TsampFilterVariant=InternalTs, TsampNgainVariant=Passthrough, TsampIntegralVariant=Disabled_SignalSpec, ExternalSaturationOutDataTypeStr=Inherit: Same as second input, DerivativeSourceVariant=Disabled, InitialConditionSetting=Auto, PreIntVariant=InternalPreInt}
      mask prompts: Controller "Simulink:masks:Controller_MP"; Form "Simulink:masks:Form_MP"; TimeDomain "Simulink:masks:TimeDomain_MP"; UseExternalTs "Simulink:masks:PIDBlockInTriggeredSubsystem_MP"; SampleTime "Simulink:masks:SampleTime1ForInherited_MP"; IntegratorMethod "Simulink:masks:IntegratorMethod_MP"; FilterMethod "Simulink:masks:FilterMethod_MP"; ControllerParametersSource "Simulink:masks:Source_MP"; P "Simulink:masks:ProportionalP_MP"; I "Simulink:masks:IntegralI_MP"; UseKiTs "Simulink:masks:UseITs_MP"; D "Simulink:masks:DerivativeD_MP"; UseExternalDerivativeSource "Simulink:masks:UseExternalDerivative_MP"; N "Simulink:masks:FilterCoefficientN_MP"; UseFilter "Simulink:masks:UseFilter_MP"; TunerSelectOption "Simulink:masks:PIDAutoTuningMethodSelect_MP"; ZeroCross "Simulink:masks:EnableZerocrossingDetection_MP"; InitialConditionSource "Simulink:masks:Source_MP"; InitialConditionForIntegrator "Simulink:masks:Integrator_MP"; InitialConditionForFilter "Simulink:masks:Filter_MP"; DifferentiatorICPrevScaledInput "Simulink:masks:Differentiator_MP"; ExternalReset "Simulink:masks:ExternalReset_MP"; IgnoreLimit "Simulink:masks:IgnoreResetWhenLinearizing_MP"; TrackingMode "Simulink:masks:EnableTrackingMode_MP"; Kt "Simulink:masks:TrackingCoefficientKt_MP"; LimitOutput "Simulink:masks:LimitOutput_MP"; SatLimitsSource "Simulink:masks:Source_MP"; UpperSaturationLimit "Simulink:masks:UpperSaturationLimit_MP"; LowerSaturationLimit "Simulink:masks:LowerSaturationLimit_MP"; LinearizeAsGain "Simulink:masks:IgnoreSaturationWhenLinearizing_MP"; AntiWindupMode "Simulink:masks:AntiwindupMethod_MP"; Kb "Simulink:masks:BackcalculationCoefficientKb_MP"; LimitIntegrator "Simulink:blkprm_prompts:IntegratorLimitOutput"; UpperIntegratorSaturationLimit "Simulink:masks:UpperSaturationLimit_MP"; LowerIntegratorSaturationLimit "Simulink:masks:LowerSaturationLimit_MP"; RndMeth "Simulink:masks:IntegerRoundingMode_MP"; SaturateOnIntegerOverflow "Simulink:masks:SaturateOnIntegerOverflow_MP"; LockScale "Simulink:masks:LockDataTypeAgainstFxpTools_MP"; PGainOutDataTypeStr "Simulink:masks:PProductOutput_MP"; PProdOutDataTypeStr "Simulink:masks:PProductOutput_MP"; IGainOutDataTypeStr "Simulink:masks:IProductOutput_MP"; IProdOutDataTypeStr "Simulink:masks:IProductOutput_MP"; DGainOutDataTypeStr "Simulink:masks:DProductOutput_MP"; DProdOutDataTypeStr "Simulink:masks:DProductOutput_MP"; NGainOutDataTypeStr "Simulink:masks:NProductOutput_MP"; NProdOutDataTypeStr "Simulink:masks:NProductOutput_MP"; SumOutDataTypeStr "Simulink:masks:SumOutput_MP"; SaturationOutDataTypeStr "Simulink:masks:SaturationOutput_MP"; PParamDataTypeStr "Simulink:masks:PParameter_MP"; IParamDataTypeStr "Simulink:masks:IParameter_MP"; DParamDataTypeStr "Simulink:masks:DParameter_MP"; NParamDataTypeStr "Simulink:masks:NParameter_MP"; KbParamDataTypeStr "Simulink:masks:KbParameter_MP"; KtParamDataTypeStr "Simulink:masks:KtParameter_MP"; KbOutDataTypeStr "Simulink:masks:KbProductOutput_MP"; KtOutDataTypeStr "Simulink:masks:KtProductOutput_MP"; IntegratorOutDataTypeStr "Simulink:masks:IntegratorOutput_MP"; FilterOutDataTypeStr "Simulink:masks:FilterOutput_MP"; SumI1OutDataTypeStr "Simulink:masks:SumI1Output_MP"; SumI2OutDataTypeStr "Simulink:masks:SumI2Output_MP"; SumI3OutDataTypeStr "Simulink:masks:SumI3Output_MP"; SumI4OutDataTypeStr "Simulink:masks:SumI4Output_MP"; SumDOutDataTypeStr "Simulink:masks:SumDOutput_MP"; SumAccumDataTypeStr "Simulink:masks:AccumulatorOfSum_MP"; SumI1AccumDataTypeStr "Simulink:masks:AccumulatorOfSumI1_MP"; SumI2AccumDataTypeStr "Simulink:masks:AccumulatorOfSumI2_MP"; SumI3AccumDataTypeStr "Simulink:masks:AccumulatorOfSumI3_MP"; SumI4AccumDataTypeStr "Simulink:masks:AccumulatorOfSumI4_MP"; SumDAccumDataTypeStr "Simulink:masks:AccumulatorOfSumD_MP"; DifferentiatorOutDataTypeStr "Simulink:masks:DifferentiatorOutput_MP"; FilterDiffNumProductOutputDataTypeStr "Simulink:masks:FilterDiffNumProductOutput_MP"; FilterDiffDenProductOutputDataTypeStr "Simulink:masks:FilterDiffDenProductOutput_MP"; FilterDiffNumAccumDataTypeStr "Simulink:masks:FilterDiffNumAccumulator_MP"; FilterDiffDenAccumDataTypeStr "Simulink:masks:FilterDiffDenAccumulator_MP"; FilterDiffOutCoefDataTypeStr "Simulink:masks:FilterDiffCoefficientOutput_MP"; ReciprocalOutDataTypeStr "Simulink:masks:FilterDiffReciprocalOutput_MP"; SumDenOutDataTypeStr "Simulink:masks:FilterDiffSumDenOutput_MP"; SumNumOutDataTypeStr "Simulink:masks:FilterDiffSumNumOutput_MP"; SumDenAccumDataTypeStr "Simulink:masks:FilterDiffSumDenAccumulator_MP"; SumNumAccumDataTypeStr "Simulink:masks:FilterDiffSumNumAccumulator_MP"; DivideOutDataTypeStr "Simulink:masks:FilterDiffDivideOutput_MP"; UdiffTsProdOutDataTypeStr "Simulink:masks:UdiffTsProdOut_MP"; NTsProdOutDataTypeStr "Simulink:masks:NTsProdOut_MP"; UintegralTsProdOutDataTypeStr "Simulink:masks:UintegralTsProdOut_MP"; UngainTsProdOutDataTypeStr "Simulink:masks:UngainTsProdOut_MP"; ClampingZeroOutDataTypeStr "Simulink:masks:ClampingAlgorithmConstantZero_MP"; FilterDenConstantOutDataTypeStr "Simulink:masks:FilterCoeffDenConstant_MP"; PCopyOutDataTypeStr "Simulink:masks:PCopyConstant_MP"; NCopyOutDataTypeStr "Simulink:masks:NCopyConstant_MP"; IntegratorContinuousStateAttributes "Simulink:masks:StateNameegposition_MP"; IntegratorStateIdentifier "Simulink:masks:StateName_MP"; IntegratorStateMustResolveToSignalObject "Simulink:masks:StateNameMustResolveToSimulinkSignalObject_MP"; IntegratorRTWStateStorageClass "Simulink:masks:CodeGenerationStorageClass_MP"; IntegratorRTWStateStorageTypeQualifier "Simulink:masks:CodeGenerationStorageTypeQualifier_MP"; FilterContinuousStateAttributes "Simulink:masks:StateNameegposition_MP"; FilterStateIdentifier "Simulink:masks:StateName_MP"; FilterStateMustResolveToSignalObject "Simulink:masks:StateNameMustResolveToSimulinkSignalObject_MP"; FilterRTWStateStorageClass "Simulink:masks:CodeGenerationStorageClass_MP"; FilterRTWStateStorageTypeQualifier "Simulink:masks:CodeGenerationStorageTypeQualifier_MP"; ParallelPVariant "Simulink:blkprm_prompts:OverrideUsingVariant"; IdealPVariant "Simulink:blkprm_prompts:OverrideUsingVariant"; IVariant "Simulink:blkprm_prompts:OverrideUsingVariant"; DVariant "Simulink:blkprm_prompts:OverrideUsingVariant"; IntegratorVariant "Simulink:blkprm_prompts:OverrideUsingVariant"; SatVariant "Simulink:blkprm_prompts:OverrideUsingVariant"; AWVariant "Simulink:blkprm_prompts:OverrideUsingVariant"; PCopyVariant "Simulink:blkprm_prompts:OverrideUsingVariant"; TRVariant "Simulink:blkprm_prompts:OverrideUsingVariant"; FdbkBlocksVariant "Simulink:blkprm_prompts:OverrideUsingVariant"; IdealPFdbkVariant "Simulink:blkprm_prompts:OverrideUsingVariant"; SatFdbkVariant "Simulink:blkprm_prompts:OverrideUsingVariant"; DerivativeFilterVariant "Simulink:blkprm_prompts:OverrideUsingVariant"; NVariant "Simulink:blkprm_prompts:OverrideUsingVariant"; NCopyVariant "Simulink:blkprm_prompts:OverrideUsingVariant"; FilterICVariant "Simulink:blkprm_prompts:OverrideUsingVariant"; IntegratorICVariant "Simulink:blkprm_prompts:OverrideUsingVariant"; ExternalResetVariant "Simulink:blkprm_prompts:OverrideUsingVariant"; TRSumVariant "Simulink:blkprm_prompts:OverrideUsingVariant"; SumFdbkVariant "Simulink:blkprm_prompts:OverrideUsingVariant"; SumVariant "Simulink:blkprm_prompts:OverrideUsingVariant"; TsampFilterVariant "Simulink:Variants:LabelComboBox"; TsampNgainVariant "Simulink:Variants:LabelComboBox"; TsampIntegralVariant "Simulink:Variants:LabelComboBox"; ExternalSaturationOutDataTypeStr "Simulink:masks:SaturationOutput_MP"; DerivativeSourceVariant "Simulink:Variants:LabelComboBox"; InitialConditionSetting "Simulink:blkprm_prompts:IntegratorInitCondSetting"; PreIntVariant "Simulink:Variants:LabelComboBox"
      mask help: Simulink:masks:PID1dof_MD
      mask init:
      | SampleTime = pidpack.PIDConfig.maskInitialization(gcbh, SampleTime);
      settings: LibrarySourceBlock=mcblib/Control/Synchronous Machine/Controllers/PI Controller  DeleteFcn=pidpack.PIDConfig.utilCloseTuner(gcb)  ModelCloseFcn=pidpack.PIDConfig.utilCloseTuner(gcb)  NameChangeFcn=pidpack.PIDConfig.utilUpdateTunerName(gcb)
      mask TypeOptions Controller: Simulink:masks:PID | Simulink:masks:PI | Simulink:masks:PD | Simulink:masks:P | Simulink:masks:I
      mask Callback Controller: pidpack.PIDConfig.callbackMaskVisibilities(gcbh,'UpdateCompFormula')
      mask TypeOptions Form: Simulink:masks:Ideal | Simulink:masks:Parallel
      mask Callback Form: pidpack.PIDConfig.callbackMaskVisibilities(gcbh,'UpdateCompFormula')
      mask TypeOptions TimeDomain: Simulink:masks:ContinuousTime | Simulink:masks:DiscreteTime
      mask Callback TimeDomain: pidpack.PIDConfig.callbackMaskVisibilities(gcbh,'UpdateCompFormula')
      mask Callback UseExternalTs: pidpack.PIDConfig.callbackMaskVisibilities(gcbh)
